simulink model "final_gimbal"  (R2026b)
settings: Solver=ode23t  StopTime=10  MaxStep=max_step  RelTol=1e-4
values from neighbouring files (symbols this model uses):
  kg = SV(i,7)    [servo_dynamics.m]
  m = add_block('simulink/Signal Routing/Mux', sprintf('    [build_model.m]
  N = 0    [LiveView.m]
  s = (1 - a) * B(k, 2:7) + a * B(k+1, 2:7)    [UdpAttitudeSource.m]    (also in build_model.m = solid(mdl, name, 'servo_dummy.stl', color, pos + [90 0 90 0])
  stl = fullfile(fileparts(fileparts(mfilename('fullpath'))), 'cad', 'stl')    [LiveView.m]
undefined symbols (not defined in the file or in its folder): ant_mass, lead_s, log_dt, mount_rate, pwm_rate, q0, servo_mass, SV, t_pure, travel, X, Y, Z
libraries: sm_lib x67, nesl_utility x18
(part 1 of 2)
settings Model: Creator=ruru  LastModifiedBy=ruru
settings SimscapeCC: SimscapeLogType=all  SimscapeNominalValues="[{\"value\":\"1\",\"unit\":\"A\"},{\"value\":\"1\",\"unit\":\"bar\"},{\"value\":\"1\",\"unit\":\"cm^2\"},{\"value\":\"1\",\"unit\":\"cm^3/s\"},{\"value\":\"1\",\"unit\":\"kJ/kg\"},{\"value\":\"1\",\"unit\":\"kW\"},{\"value\":\"1\",\"unit\":\"l\"},{\"value\":\"1\",\"unit\":\"N\"},{\"value\":\"1\",\"unit\":\"N*m\"},{\"value\":\"1\",\"unit\":\"V\"},{\"value\":\"0.001\",\"unit\":\"Wb\"}]"  SimscapeUseEnergyAccounting=off
settings ExplorerConfigSet: SimMechanicsOpenEditorOnUpdate=off

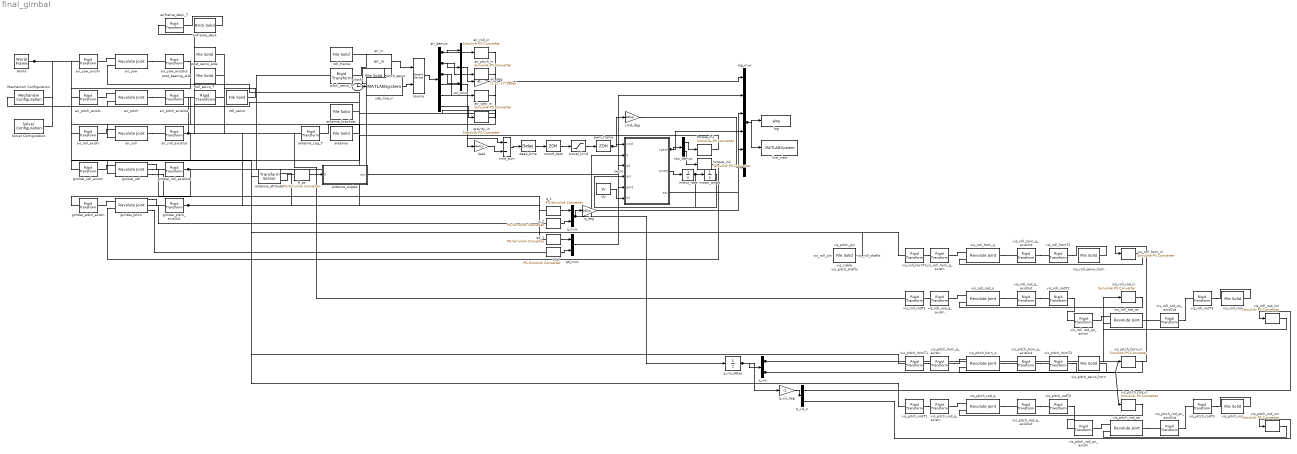
== system final_gimbal ==
  Mechanism Configuration : sm_lib/Utilities/Mechanism Configuration  UniformGravity=TimeVarying  GravityVector=[0 0 -9.80665]  GravityVectorUnits=m/s^2  LinearizationDelta=0.001  JointModeTransitionNonlinearIterations=2
  R_ps : nesl_utility/PS-Simulink Converter  PhysicalDomain=network_engine_domain  SubClassName=ps_output  LeftPortType=input  RightPortType=output  PseudoPeriodic=off  Frequencies=[]  VectorFormat=inherit  Unit=inherit  AffineConversion=off
  SV : Constant  Value=SV
  Solver Configuration : nesl_utility/Solver Configuration  PhysicalDomain=network_engine_domain  SubClassName=solver  LeftPortType=input  RightPortType=generic  Tones=[]  Harmonics=[]  SimulateNoise=off  Profile=off  UseLocalSampling=off  EnableSwitchedLinearOptims=on  FrequencyDomain=off  UseCCode=off  RelTol=0.001  AbsTol=0.001  MinStep=1e-09  ToWorkspace=off  RevertToSquareIcSolve=off  NumHomotopyIterations=100  PhasorMode=off  PhasorModeNumHarmonics=1  ConsistencySolver=NEWTON_XTOL_AFTER_FTOL  CanonicalOrdering=CANONICAL  OptimizeIntermediates=OPTIMIZED  MulticoreSolverChoice=BACKWARD_EULER  IndexReductionMethod=DerivativeReplacement  DoDC=off  ResidualTolerance=1e-09  ConsistencyTolSource=GLOBAL  ConsistencyAbsTol=0.001  ConsistencyRelTol=0.001  ConsistencyTolFactor=0.001  UseLocalSolver=off  LocalSolverChoice=NE_BACKWARD_EULER_ADVANCER  ResolveIndetEquations=on  FunctionEvalNumThread=1  LocalSolverSampleTime=0.001  DoFixedCost=off  MaxNonlinIter=3  MaxModeIter=2  ComputeImpulses=off  ImpulseIterations=2  LinearAlgebra=auto  LinearAlgebraNumThread=0  EquationFormulation=NE_TIME_EF  DelaysMemoryBudget=1024  AutomaticFiltering=on  FilteringTimeConstant=0.001  PartitionStorageMethod=AS_NEEDED  PartitionMemoryBudget=1024  PartitionMethod=BALANCED  MultibodyUseLocalSolver=off  MultibodyLocalSolverChoice=ODE1  MultibodyLocalSolverSampleTime=0.001
  World : sm_lib/Frames and Transforms/World Frame
  air_deg : Gain  Gain=[1 -1 -1]'*180/pi
  air_demux : Demux  Outputs=[1 1 1 2 2 3]
  air_in : FromWorkspace  VariableName=air_in  OutputAfterFinalValue=Holding final value
  air_mux : Mux  Inputs=3
  air_pitch : sm_lib/Joints/Revolute Joint  JointMode=Normal  CompositeWrenchDir=FollowerOnBase  CompositeWrenchFrame=BaseFrame  SenseConstraintForce=off  SenseConstraintTorque=off  SenseTotalForce=off  SenseTotalTorque=off  PositionTargetSpecify=off  PositionTargetPriority=High  PositionTargetValue=0  PositionTargetValueUnits=deg  VelocityTargetSpecify=off  VelocityTargetPriority=High  VelocityTargetValue=0  VelocityTargetValueUnits=deg/s  EquilibriumPosition=0  EquilibriumPositionUnits=deg  SpringStiffness=0  SpringStiffnessUnits=N*m/deg  DampingCoefficient=0  DampingCoefficientUnits=N*m/(deg/s)  LowerLimitSpecify=off  LowerLimitBound=-90  LowerLimitBoundUnits=deg  LowerLimitStiffness=1e4  LowerLimitStiffnessUnits=N*m/deg  LowerLimitDamping=10  LowerLimitDampingUnits=N*m/(deg/s)  LowerLimitTransitionRegionWidth=0.1  LowerLimitTransitionRegionWidthUnits=deg  UpperLimitSpecify=off  UpperLimitBound=90  UpperLimitBoundUnits=deg  UpperLimitStiffness=1e4  UpperLimitStiffnessUnits=N*m/deg  UpperLimitDamping=10  UpperLimitDampingUnits=N*m/(deg/s)  UpperLimitTransitionRegionWidth=0.1  UpperLimitTransitionRegionWidthUnits=deg  TorqueActuationMode=ComputedTorque  MotionActuationMode=InputMotion  SensePosition=off  SenseVelocity=off  SenseAcceleration=off  SenseTorqueForce=off  SenseLowerLimitTorqueForce=off  SenseUpperLimitTorqueForce=off
  air_pitch_axisIn : sm_lib/Frames and Transforms/Rigid Transform  RotationMethod=RotationMatrix  FollAlignAxisA=+X  BaseAlignAxisA=+Y  FollAlignAxisB=+Y  BaseAlignAxisB=+Z  RotationStandardAxis=+Z  RotationAngle=0  RotationAngleUnits=deg  RotationArbitraryAxis=[0 0 1]  RotationSequenceAxes=FollowerAxes  RotationSequence=XYX  RotationSequenceAngles=[0 0 0]  RotationSequenceAnglesUnits=deg  RotationMatrix=[0 1 0;0 0 1;1 0 0]  Quaternion=[1 0 0 0]  TranslationMethod=Cartesian  TranslationCartesianOffset=[0 0 0]  TranslationCartesianOffsetUnits=mm  TranslationStandardAxis=+Z  TranslationStandardOffset=0  TranslationStandardOffsetUnits=m  TranslationROffset=0  TranslationROffsetUnits=m  TranslationThetaOffset=0  TranslationThetaOffsetUnits=deg  TranslationZOffset=0  TranslationZOffsetUnits=m
  air_pitch_axisOut : sm_lib/Frames and Transforms/Rigid Transform  RotationMethod=RotationMatrix  FollAlignAxisA=+X  BaseAlignAxisA=+Y  FollAlignAxisB=+Y  BaseAlignAxisB=+Z  RotationStandardAxis=+Z  RotationAngle=0  RotationAngleUnits=deg  RotationArbitraryAxis=[0 0 1]  RotationSequenceAxes=FollowerAxes  RotationSequence=XYX  RotationSequenceAngles=[0 0 0]  RotationSequenceAnglesUnits=deg  RotationMatrix=[0 0 1;1 0 0;0 1 0]  Quaternion=[1 0 0 0]  TranslationMethod=Cartesian  TranslationCartesianOffset=[0 0 0]  TranslationCartesianOffsetUnits=mm  TranslationStandardAxis=+Z  TranslationStandardOffset=0  TranslationStandardOffsetUnits=m  TranslationROffset=0  TranslationROffsetUnits=m  TranslationThetaOffset=0  TranslationThetaOffsetUnits=deg  TranslationZOffset=0  TranslationZOffsetUnits=m
  air_pitch_in : nesl_utility/Simulink-PS Converter  PhysicalDomain=network_engine_domain  SubClassName=ps_input  LeftPortType=input  RightPortType=output  PseudoPeriodic=off  Frequencies=[]  NoiseDistribution=none  NoiseParameters=[]  Unit=rad  AffineConversion=off  FilteringAndDerivatives=filter  SimscapeFilterOrder=2  InputFilterTimeConstant=air_filter_s  UdotUserProvided=0
  air_roll : sm_lib/Joints/Revolute Joint  JointMode=Normal  CompositeWrenchDir=FollowerOnBase  CompositeWrenchFrame=BaseFrame  SenseConstraintForce=off  SenseConstraintTorque=off  SenseTotalForce=off  SenseTotalTorque=off  PositionTargetSpecify=off  PositionTargetPriority=High  PositionTargetValue=0  PositionTargetValueUnits=deg  VelocityTargetSpecify=off  VelocityTargetPriority=High  VelocityTargetValue=0  VelocityTargetValueUnits=deg/s  EquilibriumPosition=0  EquilibriumPositionUnits=deg  SpringStiffness=0  SpringStiffnessUnits=N*m/deg  DampingCoefficient=0  DampingCoefficientUnits=N*m/(deg/s)  LowerLimitSpecify=off  LowerLimitBound=-90  LowerLimitBoundUnits=deg  LowerLimitStiffness=1e4  LowerLimitStiffnessUnits=N*m/deg  LowerLimitDamping=10  LowerLimitDampingUnits=N*m/(deg/s)  LowerLimitTransitionRegionWidth=0.1  LowerLimitTransitionRegionWidthUnits=deg  UpperLimitSpecify=off  UpperLimitBound=90  UpperLimitBoundUnits=deg  UpperLimitStiffness=1e4  UpperLimitStiffnessUnits=N*m/deg  UpperLimitDamping=10  UpperLimitDampingUnits=N*m/(deg/s)  UpperLimitTransitionRegionWidth=0.1  UpperLimitTransitionRegionWidthUnits=deg  TorqueActuationMode=ComputedTorque  MotionActuationMode=InputMotion  SensePosition=off  SenseVelocity=off  SenseAcceleration=off  SenseTorqueForce=off  SenseLowerLimitTorqueForce=off  SenseUpperLimitTorqueForce=off
  air_roll_axisIn : sm_lib/Frames and Transforms/Rigid Transform  RotationMethod=RotationMatrix  FollAlignAxisA=+X  BaseAlignAxisA=+Y  FollAlignAxisB=+Y  BaseAlignAxisB=+Z  RotationStandardAxis=+Z  RotationAngle=0  RotationAngleUnits=deg  RotationArbitraryAxis=[0 0 1]  RotationSequenceAxes=FollowerAxes  RotationSequence=XYX  RotationSequenceAngles=[0 0 0]  RotationSequenceAnglesUnits=deg  RotationMatrix=[0 0 1;1 0 0;0 1 0]  Quaternion=[1 0 0 0]  TranslationMethod=Cartesian  TranslationCartesianOffset=[0 0 0]  TranslationCartesianOffsetUnits=mm  TranslationStandardAxis=+Z  TranslationStandardOffset=0  TranslationStandardOffsetUnits=m  TranslationROffset=0  TranslationROffsetUnits=m  TranslationThetaOffset=0  TranslationThetaOffsetUnits=deg  TranslationZOffset=0  TranslationZOffsetUnits=m
  air_roll_axisOut : sm_lib/Frames and Transforms/Rigid Transform  RotationMethod=RotationMatrix  FollAlignAxisA=+X  BaseAlignAxisA=+Y  FollAlignAxisB=+Y  BaseAlignAxisB=+Z  RotationStandardAxis=+Z  RotationAngle=0  RotationAngleUnits=deg  RotationArbitraryAxis=[0 0 1]  RotationSequenceAxes=FollowerAxes  RotationSequence=XYX  RotationSequenceAngles=[0 0 0]  RotationSequenceAnglesUnits=deg  RotationMatrix=[0 1 0;0 0 1;1 0 0]  Quaternion=[1 0 0 0]  TranslationMethod=Cartesian  TranslationCartesianOffset=[0 0 0]  TranslationCartesianOffsetUnits=mm  TranslationStandardAxis=+Z  TranslationStandardOffset=0  TranslationStandardOffsetUnits=m  TranslationROffset=0  TranslationROffsetUnits=m  TranslationThetaOffset=0  TranslationThetaOffsetUnits=deg  TranslationZOffset=0  TranslationZOffsetUnits=m
  air_roll_in : nesl_utility/Simulink-PS Converter  PhysicalDomain=network_engine_domain  SubClassName=ps_input  LeftPortType=input  RightPortType=output  PseudoPeriodic=off  Frequencies=[]  NoiseDistribution=none  NoiseParameters=[]  Unit=rad  AffineConversion=off  FilteringAndDerivatives=filter  SimscapeFilterOrder=2  InputFilterTimeConstant=air_filter_s  UdotUserProvided=0
  air_yaw : sm_lib/Joints/Revolute Joint  JointMode=Normal  CompositeWrenchDir=FollowerOnBase  CompositeWrenchFrame=BaseFrame  SenseConstraintForce=off  SenseConstraintTorque=off  SenseTotalForce=off  SenseTotalTorque=off  PositionTargetSpecify=off  PositionTargetPriority=High  PositionTargetValue=0  PositionTargetValueUnits=deg  VelocityTargetSpecify=off  VelocityTargetPriority=High  VelocityTargetValue=0  VelocityTargetValueUnits=deg/s  EquilibriumPosition=0  EquilibriumPositionUnits=deg  SpringStiffness=0  SpringStiffnessUnits=N*m/deg  DampingCoefficient=0  DampingCoefficientUnits=N*m/(deg/s)  LowerLimitSpecify=off  LowerLimitBound=-90  LowerLimitBoundUnits=deg  LowerLimitStiffness=1e4  LowerLimitStiffnessUnits=N*m/deg  LowerLimitDamping=10  LowerLimitDampingUnits=N*m/(deg/s)  LowerLimitTransitionRegionWidth=0.1  LowerLimitTransitionRegionWidthUnits=deg  UpperLimitSpecify=off  UpperLimitBound=90  UpperLimitBoundUnits=deg  UpperLimitStiffness=1e4  UpperLimitStiffnessUnits=N*m/deg  UpperLimitDamping=10  UpperLimitDampingUnits=N*m/(deg/s)  UpperLimitTransitionRegionWidth=0.1  UpperLimitTransitionRegionWidthUnits=deg  TorqueActuationMode=ComputedTorque  MotionActuationMode=InputMotion  SensePosition=off  SenseVelocity=off  SenseAcceleration=off  SenseTorqueForce=off  SenseLowerLimitTorqueForce=off  SenseUpperLimitTorqueForce=off
  air_yaw_axisIn : sm_lib/Frames and Transforms/Rigid Transform  RotationMethod=RotationMatrix  FollAlignAxisA=+X  BaseAlignAxisA=+Y  FollAlignAxisB=+Y  BaseAlignAxisB=+Z  RotationStandardAxis=+Z  RotationAngle=0  RotationAngleUnits=deg  RotationArbitraryAxis=[0 0 1]  RotationSequenceAxes=FollowerAxes  RotationSequence=XYX  RotationSequenceAngles=[0 0 0]  RotationSequenceAnglesUnits=deg  RotationMatrix=[1 0 0;0 1 0;0 0 1]  Quaternion=[1 0 0 0]  TranslationMethod=Cartesian  TranslationCartesianOffset=[0 0 0]  TranslationCartesianOffsetUnits=mm  TranslationStandardAxis=+Z  TranslationStandardOffset=0  TranslationStandardOffsetUnits=m  TranslationROffset=0  TranslationROffsetUnits=m  TranslationThetaOffset=0  TranslationThetaOffsetUnits=deg  TranslationZOffset=0  TranslationZOffsetUnits=m
  air_yaw_axisOut : sm_lib/Frames and Transforms/Rigid Transform  RotationMethod=RotationMatrix  FollAlignAxisA=+X  BaseAlignAxisA=+Y  FollAlignAxisB=+Y  BaseAlignAxisB=+Z  RotationStandardAxis=+Z  RotationAngle=0  RotationAngleUnits=deg  RotationArbitraryAxis=[0 0 1]  RotationSequenceAxes=FollowerAxes  RotationSequence=XYX  RotationSequenceAngles=[0 0 0]  RotationSequenceAnglesUnits=deg  RotationMatrix=[1 0 0;0 1 0;0 0 1]  Quaternion=[1 0 0 0]  TranslationMethod=Cartesian  TranslationCartesianOffset=[0 0 0]  TranslationCartesianOffsetUnits=mm  TranslationStandardAxis=+Z  TranslationStandardOffset=0  TranslationStandardOffsetUnits=m  TranslationROffset=0  TranslationROffsetUnits=m  TranslationThetaOffset=0  TranslationThetaOffsetUnits=deg  TranslationZOffset=0  TranslationZOffsetUnits=m
  air_yaw_in : nesl_utility/Simulink-PS Converter  PhysicalDomain=network_engine_domain  SubClassName=ps_input  LeftPortType=input  RightPortType=output  PseudoPeriodic=off  Frequencies=[]  NoiseDistribution=none  NoiseParameters=[]  Unit=rad  AffineConversion=off  FilteringAndDerivatives=filter  SimscapeFilterOrder=2  InputFilterTimeConstant=air_filter_s  UdotUserProvided=0
  airframe_deck : sm_lib/Body Elements/Brick Solid  BrickDimensions=[0.7 0.5 0.004]  BrickDimensionsUnits=m  ExportEntireGeometry=off  InertiaType=CalculateFromGeometry  BasedOnType=Density  Density=1000  DensityUnits=kg/m^3  Mass=1  MassUnits=kg  CenterOfMass=[0 0 0]  CenterOfMassUnits=m  MomentsOfInertia=[1 1 1]  MomentsOfInertiaUnits=kg*m^2  ProductsOfInertia=[0 0 0]  ProductsOfInertiaUnits=kg*m^2  GraphicType=FromGeometry  MarkerShape=Sphere  MarkerSize=10  GraphicVisPropType=SimpleVisualProperties  GraphicDiffuseColor=[0.8 0.8 0.78]  GraphicOpacity=1  GraphicSpecularColor=[0.5 0.5 0.5 1.0]  GraphicAmbientColor=[0.15 0.15 0.15 1.0]  GraphicEmissiveColor=[0.0 0.0 0.0 1.0]  GraphicShininess=75  DoExposeReferenceFrame=on  SerializedFrames=<Frames/>
  airframe_deck_T : sm_lib/Frames and Transforms/Rigid Transform  RotationMethod=RotationMatrix  FollAlignAxisA=+X  BaseAlignAxisA=+Y  FollAlignAxisB=+Y  BaseAlignAxisB=+Z  RotationStandardAxis=+Z  RotationAngle=0  RotationAngleUnits=deg  RotationArbitraryAxis=[0 0 1]  RotationSequenceAxes=FollowerAxes  RotationSequence=XYX  RotationSequenceAngles=[0 0 0]  RotationSequenceAnglesUnits=deg  RotationMatrix=[1 0 0;0 1 0;0 0 1]  Quaternion=[1 0 0 0]  TranslationMethod=Cartesian  TranslationCartesianOffset=[0 0 -192]  TranslationCartesianOffsetUnits=mm  TranslationStandardAxis=+Z  TranslationStandardOffset=0  TranslationStandardOffsetUnits=m  TranslationROffset=0  TranslationROffsetUnits=m  TranslationThetaOffset=0  TranslationThetaOffsetUnits=deg  TranslationZOffset=0  TranslationZOffsetUnits=m
  antenna : sm_lib/Body Elements/File Solid  ExtGeomFileName=/Users/ruru/Documenti-local/projects/hackathon/edth/hackathon-paris-2026/cad/stl/antenna_crpa_d370.stl  UnitType=Custom  ExtGeomFileUnits=mm  StepReaderType=HEX  ExportConvexHullGeometry=off  InertiaType=CalculateFromGeometry  BasedOnType=Mass  Density=1000  DensityUnits=kg/m^3  Mass=ant_mass  MassUnits=kg  CenterOfMass=[0 0 0]  CenterOfMassUnits=m  MomentsOfInertia=[1 1 1]  MomentsOfInertiaUnits=kg*m^2  ProductsOfInertia=[0 0 0]  ProductsOfInertiaUnits=kg*m^2  GraphicType=FromGeometry  MarkerShape=Sphere  MarkerSize=10  GraphicVisPropType=SimpleVisualProperties  GraphicDiffuseColor=[0.9 0.91 0.92]  GraphicOpacity=0.55  GraphicSpecularColor=[0.5 0.5 0.5 1.0]  GraphicAmbientColor=[0.15 0.15 0.15 1.0]  GraphicEmissiveColor=[0.0 0.0 0.0 1.0]  GraphicShininess=75  DoExposeReferenceFrame=on  SerializedFrames=<Frames/>
  antenna_angles : MATLAB Function  TreatAsAtomicUnit=on
  antenna_attitude : sm_lib/Frames and Transforms/Transform Sensor  ObservationFrame=World  ExpressedInFrame=World  RotationSequence=XYX  SenseAngle=off  SenseAxis=off  SenseQ=off  SenseR=on  SenseRotationSequence=off  SenseOmegaX=off  SenseOmegaY=off  SenseOmegaZ=off  SenseOmega=off  SenseQDot=off  SenseRDot=off  SenseRotationSequenceDot=off  SenseAlphaX=off  SenseAlphaY=off  SenseAlphaZ=off  SenseAlpha=off  SenseQDDot=off  SenseRDDot=off  SenseX=off  SenseY=off  SenseZ=off  SenseXYZ=off  SenseRad=off  SenseAzim=off  SenseDist=off  SenseInc=off  SenseXDot=off  SenseYDot=off  SenseZDot=off  SenseXYZDot=off  SenseRadDot=off  SenseAzimDot=off  SenseDistDot=off  SenseIncDot=off  SenseXDDot=off  SenseYDDot=off  SenseZDDot=off  SenseXYZDDot=off  SenseRadDDot=off  SenseAzimDDot=off  SenseDistDDot=off  SenseIncDDot=off
  antenna_brackets : sm_lib/Body Elements/File Solid  ExtGeomFileName=/Users/ruru/Documenti-local/projects/hackathon/edth/hackathon-paris-2026/cad/stl/antenna_brackets.stl  UnitType=Custom  ExtGeomFileUnits=mm  StepReaderType=HEX  ExportConvexHullGeometry=off  InertiaType=CalculateFromGeometry  BasedOnType=Density  Density=rho_struct  DensityUnits=kg/m^3  Mass=1  MassUnits=kg  CenterOfMass=[0 0 0]  CenterOfMassUnits=m  MomentsOfInertia=[1 1 1]  MomentsOfInertiaUnits=kg*m^2  ProductsOfInertia=[0 0 0]  ProductsOfInertiaUnits=kg*m^2  GraphicType=FromGeometry  MarkerShape=Sphere  MarkerSize=10  GraphicVisPropType=SimpleVisualProperties  GraphicDiffuseColor=[0.02 0.59 0.41]  GraphicOpacity=1  GraphicSpecularColor=[0.5 0.5 0.5 1.0]  GraphicAmbientColor=[0.15 0.15 0.15 1.0]  GraphicEmissiveColor=[0.0 0.0 0.0 1.0]  GraphicShininess=75  DoExposeReferenceFrame=on  SerializedFrames=<Frames/>
  antenna_cog_T : sm_lib/Frames and Transforms/Rigid Transform  RotationMethod=None  FollAlignAxisA=+X  BaseAlignAxisA=+Y  FollAlignAxisB=+Y  BaseAlignAxisB=+Z  RotationStandardAxis=+Z  RotationAngle=0  RotationAngleUnits=deg  RotationArbitraryAxis=[0 0 1]  RotationSequenceAxes=FollowerAxes  RotationSequence=XYX  RotationSequenceAngles=[0 0 0]  RotationSequenceAnglesUnits=deg  RotationMatrix=[1 0 0;0 1 0;0 0 1]  Quaternion=[1 0 0 0]  TranslationMethod=Cartesian  TranslationCartesianOffset=cog_offset_mm  TranslationCartesianOffsetUnits=mm  TranslationStandardAxis=+Z  TranslationStandardOffset=0  TranslationStandardOffsetUnits=m  TranslationROffset=0  TranslationROffsetUnits=m  TranslationThetaOffset=0  TranslationThetaOffsetUnits=deg  TranslationZOffset=0  TranslationZOffsetUnits=m
  clock : Clock
  cmd_deg : Gain  Gain=180/pi
  cmd_sum : Sum  Inputs=--
  dead_time : TransportDelay  DelayTime=t_pure  InitialOutput=q0
  gimbal_pitch : sm_lib/Joints/Revolute Joint  JointMode=Normal  CompositeWrenchDir=FollowerOnBase  CompositeWrenchFrame=BaseFrame  SenseConstraintForce=off  SenseConstraintTorque=off  SenseTotalForce=off  SenseTotalTorque=off  PositionTargetSpecify=on  PositionTargetPriority=High  PositionTargetValue=q0(2)  PositionTargetValueUnits=rad  VelocityTargetSpecify=off  VelocityTargetPriority=High  VelocityTargetValue=0  VelocityTargetValueUnits=deg/s  EquilibriumPosition=0  EquilibriumPositionUnits=deg  SpringStiffness=cable_k  SpringStiffnessUnits=N*m/rad  DampingCoefficient=bearing_b  DampingCoefficientUnits=N*m*s/rad  LowerLimitSpecify=off  LowerLimitBound=-90  LowerLimitBoundUnits=deg  LowerLimitStiffness=1e4  LowerLimitStiffnessUnits=N*m/deg  LowerLimitDamping=10  LowerLimitDampingUnits=N*m/(deg/s)  LowerLimitTransitionRegionWidth=0.1  LowerLimitTransitionRegionWidthUnits=deg  UpperLimitSpecify=off  UpperLimitBound=90  UpperLimitBoundUnits=deg  UpperLimitStiffness=1e4  UpperLimitStiffnessUnits=N*m/deg  UpperLimitDamping=10  UpperLimitDampingUnits=N*m/(deg/s)  UpperLimitTransitionRegionWidth=0.1  UpperLimitTransitionRegionWidthUnits=deg  TorqueActuationMode=InputTorque  MotionActuationMode=ComputedMotion  SensePosition=on  SenseVelocity=on  SenseAcceleration=off  SenseTorqueForce=off  SenseLowerLimitTorqueForce=off  SenseUpperLimitTorqueForce=off
  gimbal_pitch_axisIn : sm_lib/Frames and Transforms/Rigid Transform  RotationMethod=RotationMatrix  FollAlignAxisA=+X  BaseAlignAxisA=+Y  FollAlignAxisB=+Y  BaseAlignAxisB=+Z  RotationStandardAxis=+Z  RotationAngle=0  RotationAngleUnits=deg  RotationArbitraryAxis=[0 0 1]  RotationSequenceAxes=FollowerAxes  RotationSequence=XYX  RotationSequenceAngles=[0 0 0]  RotationSequenceAnglesUnits=deg  RotationMatrix=[0 1 0;0 0 1;1 0 0]  Quaternion=[1 0 0 0]  TranslationMethod=Cartesian  TranslationCartesianOffset=[0 0 0]  TranslationCartesianOffsetUnits=mm  TranslationStandardAxis=+Z  TranslationStandardOffset=0  TranslationStandardOffsetUnits=m  TranslationROffset=0  TranslationROffsetUnits=m  TranslationThetaOffset=0  TranslationThetaOffsetUnits=deg  TranslationZOffset=0  TranslationZOffsetUnits=m
  gimbal_pitch_axisOut : sm_lib/Frames and Transforms/Rigid Transform  RotationMethod=RotationMatrix  FollAlignAxisA=+X  BaseAlignAxisA=+Y  FollAlignAxisB=+Y  BaseAlignAxisB=+Z  RotationStandardAxis=+Z  RotationAngle=0  RotationAngleUnits=deg  RotationArbitraryAxis=[0 0 1]  RotationSequenceAxes=FollowerAxes  RotationSequence=XYX  RotationSequenceAngles=[0 0 0]  RotationSequenceAnglesUnits=deg  RotationMatrix=[0 0 1;1 0 0;0 1 0]  Quaternion=[1 0 0 0]  TranslationMethod=Cartesian  TranslationCartesianOffset=[0 0 0]  TranslationCartesianOffsetUnits=mm  TranslationStandardAxis=+Z  TranslationStandardOffset=0  TranslationStandardOffsetUnits=m  TranslationROffset=0  TranslationROffsetUnits=m  TranslationThetaOffset=0  TranslationThetaOffsetUnits=deg  TranslationZOffset=0  TranslationZOffsetUnits=m
  gimbal_roll : sm_lib/Joints/Revolute Joint  JointMode=Normal  CompositeWrenchDir=FollowerOnBase  CompositeWrenchFrame=BaseFrame  SenseConstraintForce=off  SenseConstraintTorque=off  SenseTotalForce=off  SenseTotalTorque=off  PositionTargetSpecify=on  PositionTargetPriority=High  PositionTargetValue=q0(1)  PositionTargetValueUnits=rad  VelocityTargetSpecify=off  VelocityTargetPriority=High  VelocityTargetValue=0  VelocityTargetValueUnits=deg/s  EquilibriumPosition=0  EquilibriumPositionUnits=deg  SpringStiffness=cable_k  SpringStiffnessUnits=N*m/rad  DampingCoefficient=bearing_b  DampingCoefficientUnits=N*m*s/rad  LowerLimitSpecify=off  LowerLimitBound=-90  LowerLimitBoundUnits=deg  LowerLimitStiffness=1e4  LowerLimitStiffnessUnits=N*m/deg  LowerLimitDamping=10  LowerLimitDampingUnits=N*m/(deg/s)  LowerLimitTransitionRegionWidth=0.1  LowerLimitTransitionRegionWidthUnits=deg  UpperLimitSpecify=off  UpperLimitBound=90  UpperLimitBoundUnits=deg  UpperLimitStiffness=1e4  UpperLimitStiffnessUnits=N*m/deg  UpperLimitDamping=10  UpperLimitDampingUnits=N*m/(deg/s)  UpperLimitTransitionRegionWidth=0.1  UpperLimitTransitionRegionWidthUnits=deg  TorqueActuationMode=InputTorque  MotionActuationMode=ComputedMotion  SensePosition=on  SenseVelocity=on  SenseAcceleration=off  SenseTorqueForce=off  SenseLowerLimitTorqueForce=off  SenseUpperLimitTorqueForce=off
  gimbal_roll_axisIn : sm_lib/Frames and Transforms/Rigid Transform  RotationMethod=RotationMatrix  FollAlignAxisA=+X  BaseAlignAxisA=+Y  FollAlignAxisB=+Y  BaseAlignAxisB=+Z  RotationStandardAxis=+Z  RotationAngle=0  RotationAngleUnits=deg  RotationArbitraryAxis=[0 0 1]  RotationSequenceAxes=FollowerAxes  RotationSequence=XYX  RotationSequenceAngles=[0 0 0]  RotationSequenceAnglesUnits=deg  RotationMatrix=[0 0 1;1 0 0;0 1 0]  Quaternion=[1 0 0 0]  TranslationMethod=Cartesian  TranslationCartesianOffset=[0 0 0]  TranslationCartesianOffsetUnits=mm  TranslationStandardAxis=+Z  TranslationStandardOffset=0  TranslationStandardOffsetUnits=m  TranslationROffset=0  TranslationROffsetUnits=m  TranslationThetaOffset=0  TranslationThetaOffsetUnits=deg  TranslationZOffset=0  TranslationZOffsetUnits=m
  gimbal_roll_axisOut : sm_lib/Frames and Transforms/Rigid Transform  RotationMethod=RotationMatrix  FollAlignAxisA=+X  BaseAlignAxisA=+Y  FollAlignAxisB=+Y  BaseAlignAxisB=+Z  RotationStandardAxis=+Z  RotationAngle=0  RotationAngleUnits=deg  RotationArbitraryAxis=[0 0 1]  RotationSequenceAxes=FollowerAxes  RotationSequence=XYX  RotationSequenceAngles=[0 0 0]  RotationSequenceAnglesUnits=deg  RotationMatrix=[0 1 0;0 0 1;1 0 0]  Quaternion=[1 0 0 0]  TranslationMethod=Cartesian  TranslationCartesianOffset=[0 0 0]  TranslationCartesianOffsetUnits=mm  TranslationStandardAxis=+Z  TranslationStandardOffset=0  TranslationStandardOffsetUnits=m  TranslationROffset=0  TranslationROffsetUnits=m  TranslationThetaOffset=0  TranslationThetaOffsetUnits=deg  TranslationZOffset=0  TranslationZOffsetUnits=m
  gravity_in : nesl_utility/Simulink-PS Converter  PhysicalDomain=network_engine_domain  SubClassName=ps_input  LeftPortType=input  RightPortType=output  PseudoPeriodic=off  Frequencies=[]  NoiseDistribution=none  NoiseParameters=[]  Unit=m/s^2  AffineConversion=off  FilteringAndDerivatives=provide  SimscapeFilterOrder=1  InputFilterTimeConstant=0.001  UdotUserProvided=0
  lead : Gain  Gain=lead_s
  live_view : MATLABSystem  System=LiveView  Window=20  Show=true  SimulateUsing=Interpreted execution
      mask Type: LiveView
  log : ToWorkspace  VariableName=glog  SampleTime=log_dt
  log_mux : Mux  Inputs=6
  motor_angle : Integrator  InitialCondition=q0
  motor_rate : Integrator  InitialCondition=[0;0]
  mount_task : ZeroOrderHold  SampleTime=1/mount_rate
  pitch_servo : sm_lib/Body Elements/File Solid  ExtGeomFileName=/Users/ruru/Documenti-local/projects/hackathon/edth/hackathon-paris-2026/cad/stl/servo_dummy.stl  UnitType=Custom  ExtGeomFileUnits=mm  StepReaderType=HEX  ExportConvexHullGeometry=off  InertiaType=CalculateFromGeometry  BasedOnType=Mass  Density=1000  DensityUnits=kg/m^3  Mass=servo_mass  MassUnits=kg  CenterOfMass=[0 0 0]  CenterOfMassUnits=m  MomentsOfInertia=[1 1 1]  MomentsOfInertiaUnits=kg*m^2  ProductsOfInertia=[0 0 0]  ProductsOfInertiaUnits=kg*m^2  GraphicType=FromGeometry  MarkerShape=Sphere  MarkerSize=10  GraphicVisPropType=SimpleVisualProperties  GraphicDiffuseColor=[0.12 0.16 0.22]  GraphicOpacity=1  GraphicSpecularColor=[0.5 0.5 0.5 1.0]  GraphicAmbientColor=[0.15 0.15 0.15 1.0]  GraphicEmissiveColor=[0.0 0.0 0.0 1.0]  GraphicShininess=75  DoExposeReferenceFrame=on  SerializedFrames=<Frames/>
  pitch_servo_T : sm_lib/Frames and Transforms/Rigid Transform  RotationMethod=RotationMatrix  FollAlignAxisA=+X  BaseAlignAxisA=+Y  FollAlignAxisB=+Y  BaseAlignAxisB=+Z  RotationStandardAxis=+Z  RotationAngle=0  RotationAngleUnits=deg  RotationArbitraryAxis=[0 0 1]  RotationSequenceAxes=FollowerAxes  RotationSequence=XYX  RotationSequenceAngles=[0 0 0]  RotationSequenceAnglesUnits=deg  RotationMatrix=[1 0 0;0 0 1;0 -1 0]  Quaternion=[1 0 0 0]  TranslationMethod=Cartesian  TranslationCartesianOffset=[140 189 0]  TranslationCartesianOffsetUnits=mm  TranslationStandardAxis=+Z  TranslationStandardOffset=0  TranslationStandardOffsetUnits=m  TranslationROffset=0  TranslationROffsetUnits=m  TranslationThetaOffset=0  TranslationThetaOffsetUnits=deg  TranslationZOffset=0  TranslationZOffsetUnits=m
  post_bearing_side : sm_lib/Body Elements/File Solid  ExtGeomFileName=/Users/ruru/Documenti-local/projects/hackathon/edth/hackathon-paris-2026/cad/stl/post_bearing_side.stl  UnitType=Custom  ExtGeomFileUnits=mm  StepReaderType=HEX  ExportConvexHullGeometry=off  InertiaType=CalculateFromGeometry  BasedOnType=Density  Density=rho_struct  DensityUnits=kg/m^3  Mass=1  MassUnits=kg  CenterOfMass=[0 0 0]  CenterOfMassUnits=m  MomentsOfInertia=[1 1 1]  MomentsOfInertiaUnits=kg*m^2  ProductsOfInertia=[0 0 0]  ProductsOfInertiaUnits=kg*m^2  GraphicType=FromGeometry  MarkerShape=Sphere  MarkerSize=10  GraphicVisPropType=SimpleVisualProperties  GraphicDiffuseColor=[0.42 0.45 0.5]  GraphicOpacity=1  GraphicSpecularColor=[0.5 0.5 0.5 1.0]  GraphicAmbientColor=[0.15 0.15 0.15 1.0]  GraphicEmissiveColor=[0.0 0.0 0.0 1.0]  GraphicShininess=75  DoExposeReferenceFrame=on  SerializedFrames=<Frames/>
  post_servo_side : sm_lib/Body Elements/File Solid  ExtGeomFileName=/Users/ruru/Documenti-local/projects/hackathon/edth/hackathon-paris-2026/cad/stl/post_servo_side.stl  UnitType=Custom  ExtGeomFileUnits=mm  StepReaderType=HEX  ExportConvexHullGeometry=off  InertiaType=CalculateFromGeometry  BasedOnType=Density  Density=rho_struct  DensityUnits=kg/m^3  Mass=1  MassUnits=kg  CenterOfMass=[0 0 0]  CenterOfMassUnits=m  MomentsOfInertia=[1 1 1]  MomentsOfInertiaUnits=kg*m^2  ProductsOfInertia=[0 0 0]  ProductsOfInertiaUnits=kg*m^2  GraphicType=FromGeometry  MarkerShape=Sphere  MarkerSize=10  GraphicVisPropType=SimpleVisualProperties  GraphicDiffuseColor=[0.42 0.45 0.5]  GraphicOpacity=1  GraphicSpecularColor=[0.5 0.5 0.5 1.0]  GraphicAmbientColor=[0.15 0.15 0.15 1.0]  GraphicEmissiveColor=[0.0 0.0 0.0 1.0]  GraphicShininess=75  DoExposeReferenceFrame=on  SerializedFrames=<Frames/>
  pwm_frame : ZeroOrderHold  SampleTime=1/pwm_rate
  q_1 : nesl_utility/PS-Simulink Converter  PhysicalDomain=network_engine_domain  SubClassName=ps_output  LeftPortType=input  RightPortType=output  PseudoPeriodic=off  Frequencies=[]  VectorFormat=inherit  Unit=rad  AffineConversion=off
  q_2 : nesl_utility/PS-Simulink Converter  PhysicalDomain=network_engine_domain  SubClassName=ps_output  LeftPortType=input  RightPortType=output  PseudoPeriodic=off  Frequencies=[]  VectorFormat=inherit  Unit=rad  AffineConversion=off
  q_deg : Gain  Gain=180/pi
  q_mux : Mux  Inputs=2
  q_vis : Demux  Outputs=2
  q_vis_delay : UnitDelay  InitialCondition=q0  SampleTime=0.005
  q_vis_n : Demux  Outputs=2
  q_vis_neg : Gain  Gain=-1
  qd_1 : nesl_utility/PS-Simulink Converter  PhysicalDomain=network_engine_domain  SubClassName=ps_output  LeftPortType=input  RightPortType=output  PseudoPeriodic=off  Frequencies=[]  VectorFormat=inherit  Unit=rad/s  AffineConversion=off
  qd_2 : nesl_utility/PS-Simulink Converter  PhysicalDomain=network_engine_domain  SubClassName=ps_output  LeftPortType=input  RightPortType=output  PseudoPeriodic=off  Frequencies=[]  VectorFormat=inherit  Unit=rad/s  AffineConversion=off
  qd_mux : Mux  Inputs=2
  roll_frame : sm_lib/Body Elements/File Solid  ExtGeomFileName=/Users/ruru/Documenti-local/projects/hackathon/edth/hackathon-paris-2026/cad/stl/roll_frame.stl  UnitType=Custom  ExtGeomFileUnits=mm  StepReaderType=HEX  ExportConvexHullGeometry=off  InertiaType=CalculateFromGeometry  BasedOnType=Density  Density=rho_struct  DensityUnits=kg/m^3  Mass=1  MassUnits=kg  CenterOfMass=[0 0 0]  CenterOfMassUnits=m  MomentsOfInertia=[1 1 1]  MomentsOfInertiaUnits=kg*m^2  ProductsOfInertia=[0 0 0]  ProductsOfInertiaUnits=kg*m^2  GraphicType=FromGeometry  MarkerShape=Sphere  MarkerSize=10  GraphicVisPropType=SimpleVisualProperties  GraphicDiffuseColor=[0.15 0.39 0.92]  GraphicOpacity=1  GraphicSpecularColor=[0.5 0.5 0.5 1.0]  GraphicAmbientColor=[0.15 0.15 0.15 1.0]  GraphicEmissiveColor=[0.0 0.0 0.0 1.0]  GraphicShininess=75  DoExposeReferenceFrame=on  SerializedFrames=<Frames/>
  roll_servo : sm_lib/Body Elements/File Solid  ExtGeomFileName=/Users/ruru/Documenti-local/projects/hackathon/edth/hackathon-paris-2026/cad/stl/servo_dummy.stl  UnitType=Custom  ExtGeomFileUnits=mm  StepReaderType=HEX  ExportConvexHullGeometry=off  InertiaType=CalculateFromGeometry  BasedOnType=Mass  Density=1000  DensityUnits=kg/m^3  Mass=servo_mass  MassUnits=kg  CenterOfMass=[0 0 0]  CenterOfMassUnits=m  MomentsOfInertia=[1 1 1]  MomentsOfInertiaUnits=kg*m^2  ProductsOfInertia=[0 0 0]  ProductsOfInertiaUnits=kg*m^2  GraphicType=FromGeometry  MarkerShape=Sphere  MarkerSize=10  GraphicVisPropType=SimpleVisualProperties  GraphicDiffuseColor=[0.12 0.16 0.22]  GraphicOpacity=1  GraphicSpecularColor=[0.5 0.5 0.5 1.0]  GraphicAmbientColor=[0.15 0.15 0.15 1.0]  GraphicEmissiveColor=[0.0 0.0 0.0 1.0]  GraphicShininess=75  DoExposeReferenceFrame=on  SerializedFrames=<Frames/>
  roll_servo_T : sm_lib/Frames and Transforms/Rigid Transform  RotationMethod=RotationMatrix  FollAlignAxisA=+X  BaseAlignAxisA=+Y  FollAlignAxisB=+Y  BaseAlignAxisB=+Z  RotationStandardAxis=+Z  RotationAngle=0  RotationAngleUnits=deg  RotationArbitraryAxis=[0 0 1]  RotationSequenceAxes=FollowerAxes  RotationSequence=XYX  RotationSequenceAngles=[0 0 0]  RotationSequenceAnglesUnits=deg  RotationMatrix=[0 0 1;0 1 0;-1 0 0]  Quaternion=[1 0 0 0]  TranslationMethod=Cartesian  TranslationCartesianOffset=[188 0 -127]  TranslationCartesianOffsetUnits=mm  TranslationStandardAxis=+Z  TranslationStandardOffset=0  TranslationStandardOffsetUnits=m  TranslationROffset=0  TranslationROffsetUnits=m  TranslationThetaOffset=0  TranslationThetaOffsetUnits=deg  TranslationZOffset=0  TranslationZOffsetUnits=m
  servo : MATLAB Function  TreatAsAtomicUnit=on
  source : VariantSource  VariantControls={LIVE==0, LIVE==1}
  tau_demux : Demux  Outputs=2
  torque_in1 : nesl_utility/Simulink-PS Converter  PhysicalDomain=network_engine_domain  SubClassName=ps_input  LeftPortType=input  RightPortType=output  PseudoPeriodic=off  Frequencies=[]  NoiseDistribution=none  NoiseParameters=[]  Unit=N*m  AffineConversion=off  FilteringAndDerivatives=provide  SimscapeFilterOrder=1  InputFilterTimeConstant=0.001  UdotUserProvided=0
  torque_in2 : nesl_utility/Simulink-PS Converter  PhysicalDomain=network_engine_domain  SubClassName=ps_input  LeftPortType=input  RightPortType=output  PseudoPeriodic=off  Frequencies=[]  NoiseDistribution=none  NoiseParameters=[]  Unit=N*m  AffineConversion=off  FilteringAndDerivatives=provide  SimscapeFilterOrder=1  InputFilterTimeConstant=0.001  UdotUserProvided=0
  travel_limit : Saturate  UpperLimit=travel  LowerLimit=-travel
  udp_live_in : MATLABSystem  System=UdpAttitudeSource  Port=9870  Lag=0.06  SimulateUsing=Interpreted execution
      mask Type: UdpAttitudeSource
  vis_cable : sm_lib/Body Elements/File Solid  ExtGeomFileName=/Users/ruru/Documenti-local/projects/hackathon/edth/hackathon-paris-2026/cad/stl/cable_dummy.stl  UnitType=Custom  ExtGeomFileUnits=mm  StepReaderType=HEX  ExportConvexHullGeometry=off  InertiaType=CalculateFromGeometry  BasedOnType=Mass  Density=1000  DensityUnits=kg/m^3  Mass=1e-6  MassUnits=kg  CenterOfMass=[0 0 0]  CenterOfMassUnits=m  MomentsOfInertia=[1 1 1]  MomentsOfInertiaUnits=kg*m^2  ProductsOfInertia=[0 0 0]  ProductsOfInertiaUnits=kg*m^2  GraphicType=FromGeometry  MarkerShape=Sphere  MarkerSize=10  GraphicVisPropType=SimpleVisualProperties  GraphicDiffuseColor=[0.49 0.23 0.93]  GraphicOpacity=1  GraphicSpecularColor=[0.5 0.5 0.5 1.0]  GraphicAmbientColor=[0.15 0.15 0.15 1.0]  GraphicEmissiveColor=[0.0 0.0 0.0 1.0]  GraphicShininess=75  DoExposeReferenceFrame=on  SerializedFrames=<Frames/>
  vis_pitch_hornT1 : sm_lib/Frames and Transforms/Rigid Transform  RotationMethod=RotationMatrix  FollAlignAxisA=+X  BaseAlignAxisA=+Y  FollAlignAxisB=+Y  BaseAlignAxisB=+Z  RotationStandardAxis=+Z  RotationAngle=0  RotationAngleUnits=deg  RotationArbitraryAxis=[0 0 1]  RotationSequenceAxes=FollowerAxes  RotationSequence=XYX  RotationSequenceAngles=[0 0 0]  RotationSequenceAnglesUnits=deg  RotationMatrix=[1 0 0;0 1 0;0 0 1]  Quaternion=[1 0 0 0]  TranslationMethod=Cartesian  TranslationCartesianOffset=[140 0 0]  TranslationCartesianOffsetUnits=mm  TranslationStandardAxis=+Z  TranslationStandardOffset=0  TranslationStandardOffsetUnits=m  TranslationROffset=0  TranslationROffsetUnits=m  TranslationThetaOffset=0  TranslationThetaOffsetUnits=deg  TranslationZOffset=0  TranslationZOffsetUnits=m
  vis_pitch_hornT2 : sm_lib/Frames and Transforms/Rigid Transform  RotationMethod=RotationMatrix  FollAlignAxisA=+X  BaseAlignAxisA=+Y  FollAlignAxisB=+Y  BaseAlignAxisB=+Z  RotationStandardAxis=+Z  RotationAngle=0  RotationAngleUnits=deg  RotationArbitraryAxis=[0 0 1]  RotationSequenceAxes=FollowerAxes  RotationSequence=XYX  RotationSequenceAngles=[0 0 0]  RotationSequenceAnglesUnits=deg  RotationMatrix=[1 0 0;0 1 0;0 0 1]  Quaternion=[1 0 0 0]  TranslationMethod=Cartesian  TranslationCartesianOffset=[-140 0 0]  TranslationCartesianOffsetUnits=mm  TranslationStandardAxis=+Z  TranslationStandardOffset=0  TranslationStandardOffsetUnits=m  TranslationROffset=0  TranslationROffsetUnits=m  TranslationThetaOffset=0  TranslationThetaOffsetUnits=deg  TranslationZOffset=0  TranslationZOffsetUnits=m
  vis_pitch_horn_in : nesl_utility/Simulink-PS Converter  PhysicalDomain=network_engine_domain  SubClassName=ps_input  LeftPortType=input  RightPortType=output  PseudoPeriodic=off  Frequencies=[]  NoiseDistribution=none  NoiseParameters=[]  Unit=rad  AffineConversion=off  FilteringAndDerivatives=filter  SimscapeFilterOrder=2  InputFilterTimeConstant=air_filter_s  UdotUserProvided=0
  vis_pitch_horn_q : sm_lib/Joints/Revolute Joint  JointMode=Normal  CompositeWrenchDir=FollowerOnBase  CompositeWrenchFrame=BaseFrame  SenseConstraintForce=off  SenseConstraintTorque=off  SenseTotalForce=off  SenseTotalTorque=off  PositionTargetSpecify=off  PositionTargetPriority=High  PositionTargetValue=0  PositionTargetValueUnits=deg  VelocityTargetSpecify=off  VelocityTargetPriority=High  VelocityTargetValue=0  VelocityTargetValueUnits=deg/s  EquilibriumPosition=0  EquilibriumPositionUnits=deg  SpringStiffness=0  SpringStiffnessUnits=N*m/deg  DampingCoefficient=0  DampingCoefficientUnits=N*m/(deg/s)  LowerLimitSpecify=off  LowerLimitBound=-90  LowerLimitBoundUnits=deg  LowerLimitStiffness=1e4  LowerLimitStiffnessUnits=N*m/deg  LowerLimitDamping=10  LowerLimitDampingUnits=N*m/(deg/s)  LowerLimitTransitionRegionWidth=0.1  LowerLimitTransitionRegionWidthUnits=deg  UpperLimitSpecify=off  UpperLimitBound=90  UpperLimitBoundUnits=deg  UpperLimitStiffness=1e4  UpperLimitStiffnessUnits=N*m/deg  UpperLimitDamping=10  UpperLimitDampingUnits=N*m/(deg/s)  UpperLimitTransitionRegionWidth=0.1  UpperLimitTransitionRegionWidthUnits=deg  TorqueActuationMode=ComputedTorque  MotionActuationMode=InputMotion  SensePosition=off  SenseVelocity=off  SenseAcceleration=off  SenseTorqueForce=off  SenseLowerLimitTorqueForce=off  SenseUpperLimitTorqueForce=off
  vis_pitch_horn_q_axisIn : sm_lib/Frames and Transforms/Rigid Transform  RotationMethod=RotationMatrix  FollAlignAxisA=+X  BaseAlignAxisA=+Y  FollAlignAxisB=+Y  BaseAlignAxisB=+Z  RotationStandardAxis=+Z  RotationAngle=0  RotationAngleUnits=deg  RotationArbitraryAxis=[0 0 1]  RotationSequenceAxes=FollowerAxes  RotationSequence=XYX  RotationSequenceAngles=[0 0 0]  RotationSequenceAnglesUnits=deg  RotationMatrix=[0 1 0;0 0 1;1 0 0]  Quaternion=[1 0 0 0]  TranslationMethod=Cartesian  TranslationCartesianOffset=[0 0 0]  TranslationCartesianOffsetUnits=mm  TranslationStandardAxis=+Z  TranslationStandardOffset=0  TranslationStandardOffsetUnits=m  TranslationROffset=0  TranslationROffsetUnits=m  TranslationThetaOffset=0  TranslationThetaOffsetUnits=deg  TranslationZOffset=0  TranslationZOffsetUnits=m
  vis_pitch_horn_q_axisOut : sm_lib/Frames and Transforms/Rigid Transform  RotationMethod=RotationMatrix  FollAlignAxisA=+X  BaseAlignAxisA=+Y  FollAlignAxisB=+Y  BaseAlignAxisB=+Z  RotationStandardAxis=+Z  RotationAngle=0  RotationAngleUnits=deg  RotationArbitraryAxis=[0 0 1]  RotationSequenceAxes=FollowerAxes  RotationSequence=XYX  RotationSequenceAngles=[0 0 0]  RotationSequenceAnglesUnits=deg  RotationMatrix=[0 0 1;1 0 0;0 1 0]  Quaternion=[1 0 0 0]  TranslationMethod=Cartesian  TranslationCartesianOffset=[0 0 0]  TranslationCartesianOffsetUnits=mm  TranslationStandardAxis=+Z  TranslationStandardOffset=0  TranslationStandardOffsetUnits=m  TranslationROffset=0  TranslationROffsetUnits=m  TranslationThetaOffset=0  TranslationThetaOffsetUnits=deg  TranslationZOffset=0  TranslationZOffsetUnits=m
  vis_pitch_pin : sm_lib/Body Elements/File Solid  ExtGeomFileName=/Users/ruru/Documenti-local/projects/hackathon/edth/hackathon-paris-2026/cad/stl/vis_pitch_pin.stl  UnitType=Custom  ExtGeomFileUnits=mm  StepReaderType=HEX  ExportConvexHullGeometry=off  InertiaType=CalculateFromGeometry  BasedOnType=Mass  Density=1000  DensityUnits=kg/m^3  Mass=1e-6  MassUnits=kg  CenterOfMass=[0 0 0]  CenterOfMassUnits=m  MomentsOfInertia=[1 1 1]  MomentsOfInertiaUnits=kg*m^2  ProductsOfInertia=[0 0 0]  ProductsOfInertiaUnits=kg*m^2  GraphicType=FromGeometry  MarkerShape=Sphere  MarkerSize=10  GraphicVisPropType=SimpleVisualProperties  GraphicDiffuseColor=[0.61 0.64 0.69]  GraphicOpacity=1  GraphicSpecularColor=[0.5 0.5 0.5 1.0]  GraphicAmbientColor=[0.15 0.15 0.15 1.0]  GraphicEmissiveColor=[0.0 0.0 0.0 1.0]  GraphicShininess=75  DoExposeReferenceFrame=on  SerializedFrames=<Frames/>
  vis_pitch_rod : sm_lib/Body Elements/File Solid  ExtGeomFileName=/Users/ruru/Documenti-local/projects/hackathon/edth/hackathon-paris-2026/cad/stl/vis_pitch_rod.stl  UnitType=Custom  ExtGeomFileUnits=mm  StepReaderType=HEX  ExportConvexHullGeometry=off  InertiaType=CalculateFromGeometry  BasedOnType=Mass  Density=1000  DensityUnits=kg/m^3  Mass=1e-6  MassUnits=kg  CenterOfMass=[0 0 0]  CenterOfMassUnits=m  MomentsOfInertia=[1 1 1]  MomentsOfInertiaUnits=kg*m^2  ProductsOfInertia=[0 0 0]  ProductsOfInertiaUnits=kg*m^2  GraphicType=FromGeometry  MarkerShape=Sphere  MarkerSize=10  GraphicVisPropType=SimpleVisualProperties  GraphicDiffuseColor=[0.85 0.47 0.02]  GraphicOpacity=1  GraphicSpecularColor=[0.5 0.5 0.5 1.0]  GraphicAmbientColor=[0.15 0.15 0.15 1.0]  GraphicEmissiveColor=[0.0 0.0 0.0 1.0]  GraphicShininess=75  DoExposeReferenceFrame=on  SerializedFrames=<Frames/>
  vis_pitch_rodT1 : sm_lib/Frames and Transforms/Rigid Transform  RotationMethod=RotationMatrix  FollAlignAxisA=+X  BaseAlignAxisA=+Y  FollAlignAxisB=+Y  BaseAlignAxisB=+Z  RotationStandardAxis=+Z  RotationAngle=0  RotationAngleUnits=deg  RotationArbitraryAxis=[0 0 1]  RotationSequenceAxes=FollowerAxes  RotationSequence=XYX  RotationSequenceAngles=[0 0 0]  RotationSequenceAnglesUnits=deg  RotationMatrix=[1 0 0;0 1 0;0 0 1]  Quaternion=[1 0 0 0]  TranslationMethod=Cartesian  TranslationCartesianOffset=[140 0 0]  TranslationCartesianOffsetUnits=mm  TranslationStandardAxis=+Z  TranslationStandardOffset=0  TranslationStandardOffsetUnits=m  TranslationROffset=0  TranslationROffsetUnits=m  TranslationThetaOffset=0  TranslationThetaOffsetUnits=deg  TranslationZOffset=0  TranslationZOffsetUnits=m
  vis_pitch_rodT2 : sm_lib/Frames and Transforms/Rigid Transform  RotationMethod=RotationMatrix  FollAlignAxisA=+X  BaseAlignAxisA=+Y  FollAlignAxisB=+Y  BaseAlignAxisB=+Z  RotationStandardAxis=+Z  RotationAngle=0  RotationAngleUnits=deg  RotationArbitraryAxis=[0 0 1]  RotationSequenceAxes=FollowerAxes  RotationSequence=XYX  RotationSequenceAngles=[0 0 0]  RotationSequenceAnglesUnits=deg  RotationMatrix=[1 0 0;0 1 0;0 0 1]  Quaternion=[1 0 0 0]  TranslationMethod=Cartesian  TranslationCartesianOffset=[0 0 35]  TranslationCartesianOffsetUnits=mm  TranslationStandardAxis=+Z  TranslationStandardOffset=0  TranslationStandardOffsetUnits=m  TranslationROffset=0  TranslationROffsetUnits=m  TranslationThetaOffset=0  TranslationThetaOffsetUnits=deg  TranslationZOffset=0  TranslationZOffsetUnits=m
  vis_pitch_rodT3 : sm_lib/Frames and Transforms/Rigid Transform  RotationMethod=RotationMatrix  FollAlignAxisA=+X  BaseAlignAxisA=+Y  FollAlignAxisB=+Y  BaseAlignAxisB=+Z  RotationStandardAxis=+Z  RotationAngle=0  RotationAngleUnits=deg  RotationArbitraryAxis=[0 0 1]  RotationSequenceAxes=FollowerAxes  RotationSequence=XYX  RotationSequenceAngles=[0 0 0]  RotationSequenceAnglesUnits=deg  RotationMatrix=[1 0 0;0 1 0;0 0 1]  Quaternion=[1 0 0 0]  TranslationMethod=Cartesian  TranslationCartesianOffset=[-140 0 -35]  TranslationCartesianOffsetUnits=mm  TranslationStandardAxis=+Z  TranslationStandardOffset=0  TranslationStandardOffsetUnits=m  TranslationROffset=0  TranslationROffsetUnits=m  TranslationThetaOffset=0  TranslationThetaOffsetUnits=deg  TranslationZOffset=0  TranslationZOffsetUnits=m
  vis_pitch_rod_in : nesl_utility/Simulink-PS Converter  PhysicalDomain=network_engine_domain  SubClassName=ps_input  LeftPortType=input  RightPortType=output  PseudoPeriodic=off  Frequencies=[]  NoiseDistribution=none  NoiseParameters=[]  Unit=rad  AffineConversion=off  FilteringAndDerivatives=filter  SimscapeFilterOrder=2  InputFilterTimeConstant=air_filter_s  UdotUserProvided=0
  vis_pitch_rod_inn : nesl_utility/Simulink-PS Converter  PhysicalDomain=network_engine_domain  SubClassName=ps_input  LeftPortType=input  RightPortType=output  PseudoPeriodic=off  Frequencies=[]  NoiseDistribution=none  NoiseParameters=[]  Unit=rad  AffineConversion=off  FilteringAndDerivatives=filter  SimscapeFilterOrder=2  InputFilterTimeConstant=air_filter_s  UdotUserProvided=0
  vis_pitch_rod_q : sm_lib/Joints/Revolute Joint  JointMode=Normal  CompositeWrenchDir=FollowerOnBase  CompositeWrenchFrame=BaseFrame  SenseConstraintForce=off  SenseConstraintTorque=off  SenseTotalForce=off  SenseTotalTorque=off  PositionTargetSpecify=off  PositionTargetPriority=High  PositionTargetValue=0  PositionTargetValueUnits=deg  VelocityTargetSpecify=off  VelocityTargetPriority=High  VelocityTargetValue=0  VelocityTargetValueUnits=deg/s  EquilibriumPosition=0  EquilibriumPositionUnits=deg  SpringStiffness=0  SpringStiffnessUnits=N*m/deg  DampingCoefficient=0  DampingCoefficientUnits=N*m/(deg/s)  LowerLimitSpecify=off  LowerLimitBound=-90  LowerLimitBoundUnits=deg  LowerLimitStiffness=1e4  LowerLimitStiffnessUnits=N*m/deg  LowerLimitDamping=10  LowerLimitDampingUnits=N*m/(deg/s)  LowerLimitTransitionRegionWidth=0.1  LowerLimitTransitionRegionWidthUnits=deg  UpperLimitSpecify=off  UpperLimitBound=90  UpperLimitBoundUnits=deg  UpperLimitStiffness=1e4  UpperLimitStiffnessUnits=N*m/deg  UpperLimitDamping=10  UpperLimitDampingUnits=N*m/(deg/s)  UpperLimitTransitionRegionWidth=0.1  UpperLimitTransitionRegionWidthUnits=deg  TorqueActuationMode=ComputedTorque  MotionActuationMode=InputMotion  SensePosition=off  SenseVelocity=off  SenseAcceleration=off  SenseTorqueForce=off  SenseLowerLimitTorqueForce=off  SenseUpperLimitTorqueForce=off
  vis_pitch_rod_q_axisIn : sm_lib/Frames and Transforms/Rigid Transform  RotationMethod=RotationMatrix  FollAlignAxisA=+X  BaseAlignAxisA=+Y  FollAlignAxisB=+Y  BaseAlignAxisB=+Z  RotationStandardAxis=+Z  RotationAngle=0  RotationAngleUnits=deg  RotationArbitraryAxis=[0 0 1]  RotationSequenceAxes=FollowerAxes  RotationSequence=XYX  RotationSequenceAngles=[0 0 0]  RotationSequenceAnglesUnits=deg  RotationMatrix=[0 1 0;0 0 1;1 0 0]  Quaternion=[1 0 0 0]  TranslationMethod=Cartesian  TranslationCartesianOffset=[0 0 0]  TranslationCartesianOffsetUnits=mm  TranslationStandardAxis=+Z  TranslationStandardOffset=0  TranslationStandardOffsetUnits=m  TranslationROffset=0  TranslationROffsetUnits=m  TranslationThetaOffset=0  TranslationThetaOffsetUnits=deg  TranslationZOffset=0  TranslationZOffsetUnits=m
  vis_pitch_rod_q_axisOut : sm_lib/Frames and Transforms/Rigid Transform  RotationMethod=RotationMatrix  FollAlignAxisA=+X  BaseAlignAxisA=+Y  FollAlignAxisB=+Y  BaseAlignAxisB=+Z  RotationStandardAxis=+Z  RotationAngle=0  RotationAngleUnits=deg  RotationArbitraryAxis=[0 0 1]  RotationSequenceAxes=FollowerAxes  RotationSequence=XYX  RotationSequenceAngles=[0 0 0]  RotationSequenceAnglesUnits=deg  RotationMatrix=[0 0 1;1 0 0;0 1 0]  Quaternion=[1 0 0 0]  TranslationMethod=Cartesian  TranslationCartesianOffset=[0 0 0]  TranslationCartesianOffsetUnits=mm  TranslationStandardAxis=+Z  TranslationStandardOffset=0  TranslationStandardOffsetUnits=m  TranslationROffset=0  TranslationROffsetUnits=m  TranslationThetaOffset=0  TranslationThetaOffsetUnits=deg  TranslationZOffset=0  TranslationZOffsetUnits=m
  vis_pitch_rod_qn : sm_lib/Joints/Revolute Joint  JointMode=Normal  CompositeWrenchDir=FollowerOnBase  CompositeWrenchFrame=BaseFrame  SenseConstraintForce=off  SenseConstraintTorque=off  SenseTotalForce=off  SenseTotalTorque=off  PositionTargetSpecify=off  PositionTargetPriority=High  PositionTargetValue=0  PositionTargetValueUnits=deg  VelocityTargetSpecify=off  VelocityTargetPriority=High  VelocityTargetValue=0  VelocityTargetValueUnits=deg/s  EquilibriumPosition=0  EquilibriumPositionUnits=deg  SpringStiffness=0  SpringStiffnessUnits=N*m/deg  DampingCoefficient=0  DampingCoefficientUnits=N*m/(deg/s)  LowerLimitSpecify=off  LowerLimitBound=-90  LowerLimitBoundUnits=deg  LowerLimitStiffness=1e4  LowerLimitStiffnessUnits=N*m/deg  LowerLimitDamping=10  LowerLimitDampingUnits=N*m/(deg/s)  LowerLimitTransitionRegionWidth=0.1  LowerLimitTransitionRegionWidthUnits=deg  UpperLimitSpecify=off  UpperLimitBound=90  UpperLimitBoundUnits=deg  UpperLimitStiffness=1e4  UpperLimitStiffnessUnits=N*m/deg  UpperLimitDamping=10  UpperLimitDampingUnits=N*m/(deg/s)  UpperLimitTransitionRegionWidth=0.1  UpperLimitTransitionRegionWidthUnits=deg  TorqueActuationMode=ComputedTorque  MotionActuationMode=InputMotion  SensePosition=off  SenseVelocity=off  SenseAcceleration=off  SenseTorqueForce=off  SenseLowerLimitTorqueForce=off  SenseUpperLimitTorqueForce=off
  vis_pitch_rod_qn_axisIn : sm_lib/Frames and Transforms/Rigid Transform  RotationMethod=RotationMatrix  FollAlignAxisA=+X  BaseAlignAxisA=+Y  FollAlignAxisB=+Y  BaseAlignAxisB=+Z  RotationStandardAxis=+Z  RotationAngle=0  RotationAngleUnits=deg  RotationArbitraryAxis=[0 0 1]  RotationSequenceAxes=FollowerAxes  RotationSequence=XYX  RotationSequenceAngles=[0 0 0]  RotationSequenceAnglesUnits=deg  RotationMatrix=[0 1 0;0 0 1;1 0 0]  Quaternion=[1 0 0 0]  TranslationMethod=Cartesian  TranslationCartesianOffset=[0 0 0]  TranslationCartesianOffsetUnits=mm  TranslationStandardAxis=+Z  TranslationStandardOffset=0  TranslationStandardOffsetUnits=m  TranslationROffset=0  TranslationROffsetUnits=m  TranslationThetaOffset=0  TranslationThetaOffsetUnits=deg  TranslationZOffset=0  TranslationZOffsetUnits=m
  vis_pitch_rod_qn_axisOut : sm_lib/Frames and Transforms/Rigid Transform  RotationMethod=RotationMatrix  FollAlignAxisA=+X  BaseAlignAxisA=+Y  FollAlignAxisB=+Y  BaseAlignAxisB=+Z  RotationStandardAxis=+Z  RotationAngle=0  RotationAngleUnits=deg  RotationArbitraryAxis=[0 0 1]  RotationSequenceAxes=FollowerAxes  RotationSequence=XYX  RotationSequenceAngles=[0 0 0]  RotationSequenceAnglesUnits=deg  RotationMatrix=[0 0 1;1 0 0;0 1 0]  Quaternion=[1 0 0 0]  TranslationMethod=Cartesian  TranslationCartesianOffset=[0 0 0]  TranslationCartesianOffsetUnits=mm  TranslationStandardAxis=+Z  TranslationStandardOffset=0  TranslationStandardOffsetUnits=m  TranslationROffset=0  TranslationROffsetUnits=m  TranslationThetaOffset=0  TranslationThetaOffsetUnits=deg  TranslationZOffset=0  TranslationZOffsetUnits=m
  vis_pitch_servo_horn : sm_lib/Body Elements/File Solid  ExtGeomFileName=/Users/ruru/Documenti-local/projects/hackathon/edth/hackathon-paris-2026/cad/stl/vis_pitch_servo_horn.stl  UnitType=Custom  ExtGeomFileUnits=mm  StepReaderType=HEX  ExportConvexHullGeometry=off  InertiaType=CalculateFromGeometry  BasedOnType=Mass  Density=1000  DensityUnits=kg/m^3  Mass=1e-6  MassUnits=kg  CenterOfMass=[0 0 0]  CenterOfMassUnits=m  MomentsOfInertia=[1 1 1]  MomentsOfInertiaUnits=kg*m^2  ProductsOfInertia=[0 0 0]  ProductsOfInertiaUnits=kg*m^2  GraphicType=FromGeometry  MarkerShape=Sphere  MarkerSize=10  GraphicVisPropType=SimpleVisualProperties  GraphicDiffuseColor=[0.85 0.47 0.02]  GraphicOpacity=1  GraphicSpecularColor=[0.5 0.5 0.5 1.0]  GraphicAmbientColor=[0.15 0.15 0.15 1.0]  GraphicEmissiveColor=[0.0 0.0 0.0 1.0]  GraphicShininess=75  DoExposeReferenceFrame=on  SerializedFrames=<Frames/>
  vis_pitch_shafts : sm_lib/Body Elements/File Solid  ExtGeomFileName=/Users/ruru/Documenti-local/projects/hackathon/edth/hackathon-paris-2026/cad/stl/vis_pitch_shafts.stl  UnitType=Custom  ExtGeomFileUnits=mm  StepReaderType=HEX  ExportConvexHullGeometry=off  InertiaType=CalculateFromGeometry  BasedOnType=Mass  Density=1000  DensityUnits=kg/m^3  Mass=1e-6  MassUnits=kg  CenterOfMass=[0 0 0]  CenterOfMassUnits=m  MomentsOfInertia=[1 1 1]  MomentsOfInertiaUnits=kg*m^2  ProductsOfInertia=[0 0 0]  ProductsOfInertiaUnits=kg*m^2  GraphicType=FromGeometry  MarkerShape=Sphere  MarkerSize=10  GraphicVisPropType=SimpleVisualProperties  GraphicDiffuseColor=[0.61 0.64 0.69]  GraphicOpacity=1  GraphicSpecularColor=[0.5 0.5 0.5 1.0]  GraphicAmbientColor=[0.15 0.15 0.15 1.0]  GraphicEmissiveColor=[0.0 0.0 0.0 1.0]  GraphicShininess=75  DoExposeReferenceFrame=on  SerializedFrames=<Frames/>
  vis_roll_hornT1 : sm_lib/Frames and Transforms/Rigid Transform  RotationMethod=RotationMatrix  FollAlignAxisA=+X  BaseAlignAxisA=+Y  FollAlignAxisB=+Y  BaseAlignAxisB=+Z  RotationStandardAxis=+Z  RotationAngle=0  RotationAngleUnits=deg  RotationArbitraryAxis=[0 0 1]  RotationSequenceAxes=FollowerAxes  RotationSequence=XYX  RotationSequenceAngles=[0 0 0]  RotationSequenceAnglesUnits=deg  RotationMatrix=[1 0 0;0 1 0;0 0 1]  Quaternion=[1 0 0 0]  TranslationMethod=Cartesian  TranslationCartesianOffset=[0 0 -127]  TranslationCartesianOffsetUnits=mm  TranslationStandardAxis=+Z  TranslationStandardOffset=0  TranslationStandardOffsetUnits=m  TranslationROffset=0  TranslationROffsetUnits=m  TranslationThetaOffset=0  TranslationThetaOffsetUnits=deg  TranslationZOffset=0  TranslationZOffsetUnits=m
  vis_roll_hornT2 : sm_lib/Frames and Transforms/Rigid Transform  RotationMethod=RotationMatrix  FollAlignAxisA=+X  BaseAlignAxisA=+Y  FollAlignAxisB=+Y  BaseAlignAxisB=+Z  RotationStandardAxis=+Z  RotationAngle=0  RotationAngleUnits=deg  RotationArbitraryAxis=[0 0 1]  RotationSequenceAxes=FollowerAxes  RotationSequence=XYX  RotationSequenceAngles=[0 0 0]  RotationSequenceAnglesUnits=deg  RotationMatrix=[1 0 0;0 1 0;0 0 1]  Quaternion=[1 0 0 0]  TranslationMethod=Cartesian  TranslationCartesianOffset=[0 0 127]  TranslationCartesianOffsetUnits=mm  TranslationStandardAxis=+Z  TranslationStandardOffset=0  TranslationStandardOffsetUnits=m  TranslationROffset=0  TranslationROffsetUnits=m  TranslationThetaOffset=0  TranslationThetaOffsetUnits=deg  TranslationZOffset=0  TranslationZOffsetUnits=m
  vis_roll_horn_in : nesl_utility/Simulink-PS Converter  PhysicalDomain=network_engine_domain  SubClassName=ps_input  LeftPortType=input  RightPortType=output  PseudoPeriodic=off  Frequencies=[]  NoiseDistribution=none  NoiseParameters=[]  Unit=rad  AffineConversion=off  FilteringAndDerivatives=filter  SimscapeFilterOrder=2  InputFilterTimeConstant=air_filter_s  UdotUserProvided=0
  vis_roll_horn_q : sm_lib/Joints/Revolute Joint  JointMode=Normal  CompositeWrenchDir=FollowerOnBase  CompositeWrenchFrame=BaseFrame  SenseConstraintForce=off  SenseConstraintTorque=off  SenseTotalForce=off  SenseTotalTorque=off  PositionTargetSpecify=off  PositionTargetPriority=High  PositionTargetValue=0  PositionTargetValueUnits=deg  VelocityTargetSpecify=off  VelocityTargetPriority=High  VelocityTargetValue=0  VelocityTargetValueUnits=deg/s  EquilibriumPosition=0  EquilibriumPositionUnits=deg  SpringStiffness=0  SpringStiffnessUnits=N*m/deg  DampingCoefficient=0  DampingCoefficientUnits=N*m/(deg/s)  LowerLimitSpecify=off  LowerLimitBound=-90  LowerLimitBoundUnits=deg  LowerLimitStiffness=1e4  LowerLimitStiffnessUnits=N*m/deg  LowerLimitDamping=10  LowerLimitDampingUnits=N*m/(deg/s)  LowerLimitTransitionRegionWidth=0.1  LowerLimitTransitionRegionWidthUnits=deg  UpperLimitSpecify=off  UpperLimitBound=90  UpperLimitBoundUnits=deg  UpperLimitStiffness=1e4  UpperLimitStiffnessUnits=N*m/deg  UpperLimitDamping=10  UpperLimitDampingUnits=N*m/(deg/s)  UpperLimitTransitionRegionWidth=0.1  UpperLimitTransitionRegionWidthUnits=deg  TorqueActuationMode=ComputedTorque  MotionActuationMode=InputMotion  SensePosition=off  SenseVelocity=off  SenseAcceleration=off  SenseTorqueForce=off  SenseLowerLimitTorqueForce=off  SenseUpperLimitTorqueForce=off
  vis_roll_horn_q_axisIn : sm_lib/Frames and Transforms/Rigid Transform  RotationMethod=RotationMatrix  FollAlignAxisA=+X  BaseAlignAxisA=+Y  FollAlignAxisB=+Y  BaseAlignAxisB=+Z  RotationStandardAxis=+Z  RotationAngle=0  RotationAngleUnits=deg  RotationArbitraryAxis=[0 0 1]  RotationSequenceAxes=FollowerAxes  RotationSequence=XYX  RotationSequenceAngles=[0 0 0]  RotationSequenceAnglesUnits=deg  RotationMatrix=[0 0 1;1 0 0;0 1 0]  Quaternion=[1 0 0 0]  TranslationMethod=Cartesian  TranslationCartesianOffset=[0 0 0]  TranslationCartesianOffsetUnits=mm  TranslationStandardAxis=+Z  TranslationStandardOffset=0  TranslationStandardOffsetUnits=m  TranslationROffset=0  TranslationROffsetUnits=m  TranslationThetaOffset=0  TranslationThetaOffsetUnits=deg  TranslationZOffset=0  TranslationZOffsetUnits=m
  vis_roll_horn_q_axisOut : sm_lib/Frames and Transforms/Rigid Transform  RotationMethod=RotationMatrix  FollAlignAxisA=+X  BaseAlignAxisA=+Y  FollAlignAxisB=+Y  BaseAlignAxisB=+Z  RotationStandardAxis=+Z  RotationAngle=0  RotationAngleUnits=deg  RotationArbitraryAxis=[0 0 1]  RotationSequenceAxes=FollowerAxes  RotationSequence=XYX  RotationSequenceAngles=[0 0 0]  RotationSequenceAnglesUnits=deg  RotationMatrix=[0 1 0;0 0 1;1 0 0]  Quaternion=[1 0 0 0]  TranslationMethod=Cartesian  TranslationCartesianOffset=[0 0 0]  TranslationCartesianOffsetUnits=mm  TranslationStandardAxis=+Z  TranslationStandardOffset=0  TranslationStandardOffsetUnits=m  TranslationROffset=0  TranslationROffsetUnits=m  TranslationThetaOffset=0  TranslationThetaOffsetUnits=deg  TranslationZOffset=0  TranslationZOffsetUnits=m
  vis_roll_pin : sm_lib/Body Elements/File Solid  ExtGeomFileName=/Users/ruru/Documenti-local/projects/hackathon/edth/hackathon-paris-2026/cad/stl/vis_roll_pin.stl  UnitType=Custom  ExtGeomFileUnits=mm  StepReaderType=HEX  ExportConvexHullGeometry=off  InertiaType=CalculateFromGeometry  BasedOnType=Mass  Density=1000  DensityUnits=kg/m^3  Mass=1e-6  MassUnits=kg  CenterOfMass=[0 0 0]  CenterOfMassUnits=m  MomentsOfInertia=[1 1 1]  MomentsOfInertiaUnits=kg*m^2  ProductsOfInertia=[0 0 0]  ProductsOfInertiaUnits=kg*m^2  GraphicType=FromGeometry  MarkerShape=Sphere  MarkerSize=10  GraphicVisPropType=SimpleVisualProperties  GraphicDiffuseColor=[0.61 0.64 0.69]  GraphicOpacity=1  GraphicSpecularColor=[0.5 0.5 0.5 1.0]  GraphicAmbientColor=[0.15 0.15 0.15 1.0]  GraphicEmissiveColor=[0.0 0.0 0.0 1.0]  GraphicShininess=75  DoExposeReferenceFrame=on  SerializedFrames=<Frames/>
  vis_roll_rod : sm_lib/Body Elements/File Solid  ExtGeomFileName=/Users/ruru/Documenti-local/projects/hackathon/edth/hackathon-paris-2026/cad/stl/vis_roll_rod.stl  UnitType=Custom  ExtGeomFileUnits=mm  StepReaderType=HEX  ExportConvexHullGeometry=off  InertiaType=CalculateFromGeometry  BasedOnType=Mass  Density=1000  DensityUnits=kg/m^3  Mass=1e-6  MassUnits=kg  CenterOfMass=[0 0 0]  CenterOfMassUnits=m  MomentsOfInertia=[1 1 1]  MomentsOfInertiaUnits=kg*m^2  ProductsOfInertia=[0 0 0]  ProductsOfInertiaUnits=kg*m^2  GraphicType=FromGeometry  MarkerShape=Sphere  MarkerSize=10  GraphicVisPropType=SimpleVisualProperties  GraphicDiffuseColor=[0.85 0.47 0.02]  GraphicOpacity=1  GraphicSpecularColor=[0.5 0.5 0.5 1.0]  GraphicAmbientColor=[0.15 0.15 0.15 1.0]  GraphicEmissiveColor=[0.0 0.0 0.0 1.0]  GraphicShininess=75  DoExposeReferenceFrame=on  SerializedFrames=<Frames/>
  vis_roll_rodT1 : sm_lib/Frames and Transforms/Rigid Transform  RotationMethod=RotationMatrix  FollAlignAxisA=+X  BaseAlignAxisA=+Y  FollAlignAxisB=+Y  BaseAlignAxisB=+Z  RotationStandardAxis=+Z  RotationAngle=0  RotationAngleUnits=deg  RotationArbitraryAxis=[0 0 1]  RotationSequenceAxes=FollowerAxes  RotationSequence=XYX  RotationSequenceAngles=[0 0 0]  RotationSequenceAnglesUnits=deg  RotationMatrix=[1 0 0;0 1 0;0 0 1]  Quaternion=[1 0 0 0]  TranslationMethod=Cartesian  TranslationCartesianOffset=[0 0 -127]  TranslationCartesianOffsetUnits=mm  TranslationStandardAxis=+Z  TranslationStandardOffset=0  TranslationStandardOffsetUnits=m  TranslationROffset=0  TranslationROffsetUnits=m  TranslationThetaOffset=0  TranslationThetaOffsetUnits=deg  TranslationZOffset=0  TranslationZOffsetUnits=m
  vis_roll_rodT2 : sm_lib/Frames and Transforms/Rigid Transform  RotationMethod=RotationMatrix  FollAlignAxisA=+X  BaseAlignAxisA=+Y  FollAlignAxisB=+Y  BaseAlignAxisB=+Z  RotationStandardAxis=+Z  RotationAngle=0  RotationAngleUnits=deg  RotationArbitraryAxis=[0 0 1]  RotationSequenceAxes=FollowerAxes  RotationSequence=XYX  RotationSequenceAngles=[0 0 0]  RotationSequenceAnglesUnits=deg  RotationMatrix=[1 0 0;0 1 0;0 0 1]  Quaternion=[1 0 0 0]  TranslationMethod=Cartesian  TranslationCartesianOffset=[0 25 0]  TranslationCartesianOffsetUnits=mm  TranslationStandardAxis=+Z  TranslationStandardOffset=0  TranslationStandardOffsetUnits=m  TranslationROffset=0  TranslationROffsetUnits=m  TranslationThetaOffset=0  TranslationThetaOffsetUnits=deg  TranslationZOffset=0  TranslationZOffsetUnits=m
  vis_roll_rodT3 : sm_lib/Frames and Transforms/Rigid Transform  RotationMethod=RotationMatrix  FollAlignAxisA=+X  BaseAlignAxisA=+Y  FollAlignAxisB=+Y  BaseAlignAxisB=+Z  RotationStandardAxis=+Z  RotationAngle=0  RotationAngleUnits=deg  RotationArbitraryAxis=[0 0 1]  RotationSequenceAxes=FollowerAxes  RotationSequence=XYX  RotationSequenceAngles=[0 0 0]  RotationSequenceAnglesUnits=deg  RotationMatrix=[1 0 0;0 1 0;0 0 1]  Quaternion=[1 0 0 0]  TranslationMethod=Cartesian  TranslationCartesianOffset=[0 -25 127]  TranslationCartesianOffsetUnits=mm  TranslationStandardAxis=+Z  TranslationStandardOffset=0  TranslationStandardOffsetUnits=m  TranslationROffset=0  TranslationROffsetUnits=m  TranslationThetaOffset=0  TranslationThetaOffsetUnits=deg  TranslationZOffset=0  TranslationZOffsetUnits=m
  vis_roll_rod_in : nesl_utility/Simulink-PS Converter  PhysicalDomain=network_engine_domain  SubClassName=ps_input  LeftPortType=input  RightPortType=output  PseudoPeriodic=off  Frequencies=[]  NoiseDistribution=none  NoiseParameters=[]  Unit=rad  AffineConversion=off  FilteringAndDerivatives=filter  SimscapeFilterOrder=2  InputFilterTimeConstant=air_filter_s  UdotUserProvided=0
  vis_roll_rod_inn : nesl_utility/Simulink-PS Converter  PhysicalDomain=network_engine_domain  SubClassName=ps_input  LeftPortType=input  RightPortType=output  PseudoPeriodic=off  Frequencies=[]  NoiseDistribution=none  NoiseParameters=[]  Unit=rad  AffineConversion=off  FilteringAndDerivatives=filter  SimscapeFilterOrder=2  InputFilterTimeConstant=air_filter_s  UdotUserProvided=0
  vis_roll_rod_q : sm_lib/Joints/Revolute Joint  JointMode=Normal  CompositeWrenchDir=FollowerOnBase  CompositeWrenchFrame=BaseFrame  SenseConstraintForce=off  SenseConstraintTorque=off  SenseTotalForce=off  SenseTotalTorque=off  PositionTargetSpecify=off  PositionTargetPriority=High  PositionTargetValue=0  PositionTargetValueUnits=deg  VelocityTargetSpecify=off  VelocityTargetPriority=High  VelocityTargetValue=0  VelocityTargetValueUnits=deg/s  EquilibriumPosition=0  EquilibriumPositionUnits=deg  SpringStiffness=0  SpringStiffnessUnits=N*m/deg  DampingCoefficient=0  DampingCoefficientUnits=N*m/(deg/s)  LowerLimitSpecify=off  LowerLimitBound=-90  LowerLimitBoundUnits=deg  LowerLimitStiffness=1e4  LowerLimitStiffnessUnits=N*m/deg  LowerLimitDamping=10  LowerLimitDampingUnits=N*m/(deg/s)  LowerLimitTransitionRegionWidth=0.1  LowerLimitTransitionRegionWidthUnits=deg  UpperLimitSpecify=off  UpperLimitBound=90  UpperLimitBoundUnits=deg  UpperLimitStiffness=1e4  UpperLimitStiffnessUnits=N*m/deg  UpperLimitDamping=10  UpperLimitDampingUnits=N*m/(deg/s)  UpperLimitTransitionRegionWidth=0.1  UpperLimitTransitionRegionWidthUnits=deg  TorqueActuationMode=ComputedTorque  MotionActuationMode=InputMotion  SensePosition=off  SenseVelocity=off  SenseAcceleration=off  SenseTorqueForce=off  SenseLowerLimitTorqueForce=off  SenseUpperLimitTorqueForce=off
  vis_roll_rod_q_axisIn : sm_lib/Frames and Transforms/Rigid Transform  RotationMethod=RotationMatrix  FollAlignAxisA=+X  BaseAlignAxisA=+Y  FollAlignAxisB=+Y  BaseAlignAxisB=+Z  RotationStandardAxis=+Z  RotationAngle=0  RotationAngleUnits=deg  RotationArbitraryAxis=[0 0 1]  RotationSequenceAxes=FollowerAxes  RotationSequence=XYX  RotationSequenceAngles=[0 0 0]  RotationSequenceAnglesUnits=deg  RotationMatrix=[0 0 1;1 0 0;0 1 0]  Quaternion=[1 0 0 0]  TranslationMethod=Cartesian  TranslationCartesianOffset=[0 0 0]  TranslationCartesianOffsetUnits=mm  TranslationStandardAxis=+Z  TranslationStandardOffset=0  TranslationStandardOffsetUnits=m  TranslationROffset=0  TranslationROffsetUnits=m  TranslationThetaOffset=0  TranslationThetaOffsetUnits=deg  TranslationZOffset=0  TranslationZOffsetUnits=m
  vis_roll_rod_q_axisOut : sm_lib/Frames and Transforms/Rigid Transform  RotationMethod=RotationMatrix  FollAlignAxisA=+X  BaseAlignAxisA=+Y  FollAlignAxisB=+Y  BaseAlignAxisB=+Z  RotationStandardAxis=+Z  RotationAngle=0  RotationAngleUnits=deg  RotationArbitraryAxis=[0 0 1]  RotationSequenceAxes=FollowerAxes  RotationSequence=XYX  RotationSequenceAngles=[0 0 0]  RotationSequenceAnglesUnits=deg  RotationMatrix=[0 1 0;0 0 1;1 0 0]  Quaternion=[1 0 0 0]  TranslationMethod=Cartesian  TranslationCartesianOffset=[0 0 0]  TranslationCartesianOffsetUnits=mm  TranslationStandardAxis=+Z  TranslationStandardOffset=0  TranslationStandardOffsetUnits=m  TranslationROffset=0  TranslationROffsetUnits=m  TranslationThetaOffset=0  TranslationThetaOffsetUnits=deg  TranslationZOffset=0  TranslationZOffsetUnits=m
  vis_roll_rod_qn : sm_lib/Joints/Revolute Joint  JointMode=Normal  CompositeWrenchDir=FollowerOnBase  CompositeWrenchFrame=BaseFrame  SenseConstraintForce=off  SenseConstraintTorque=off  SenseTotalForce=off  SenseTotalTorque=off  PositionTargetSpecify=off  PositionTargetPriority=High  PositionTargetValue=0  PositionTargetValueUnits=deg  VelocityTargetSpecify=off  VelocityTargetPriority=High  VelocityTargetValue=0  VelocityTargetValueUnits=deg/s  EquilibriumPosition=0  EquilibriumPositionUnits=deg  SpringStiffness=0  SpringStiffnessUnits=N*m/deg  DampingCoefficient=0  DampingCoefficientUnits=N*m/(deg/s)  LowerLimitSpecify=off  LowerLimitBound=-90  LowerLimitBoundUnits=deg  LowerLimitStiffness=1e4  LowerLimitStiffnessUnits=N*m/deg  LowerLimitDamping=10  LowerLimitDampingUnits=N*m/(deg/s)  LowerLimitTransitionRegionWidth=0.1  LowerLimitTransitionRegionWidthUnits=deg  UpperLimitSpecify=off  UpperLimitBound=90  UpperLimitBoundUnits=deg  UpperLimitStiffness=1e4  UpperLimitStiffnessUnits=N*m/deg  UpperLimitDamping=10  UpperLimitDampingUnits=N*m/(deg/s)  UpperLimitTransitionRegionWidth=0.1  UpperLimitTransitionRegionWidthUnits=deg  TorqueActuationMode=ComputedTorque  MotionActuationMode=InputMotion  SensePosition=off  SenseVelocity=off  SenseAcceleration=off  SenseTorqueForce=off  SenseLowerLimitTorqueForce=off  SenseUpperLimitTorqueForce=off
  vis_roll_rod_qn_axisIn : sm_lib/Frames and Transforms/Rigid Transform  RotationMethod=RotationMatrix  FollAlignAxisA=+X  BaseAlignAxisA=+Y  FollAlignAxisB=+Y  BaseAlignAxisB=+Z  RotationStandardAxis=+Z  RotationAngle=0  RotationAngleUnits=deg  RotationArbitraryAxis=[0 0 1]  RotationSequenceAxes=FollowerAxes  RotationSequence=XYX  RotationSequenceAngles=[0 0 0]  RotationSequenceAnglesUnits=deg  RotationMatrix=[0 0 1;1 0 0;0 1 0]  Quaternion=[1 0 0 0]  TranslationMethod=Cartesian  TranslationCartesianOffset=[0 0 0]  TranslationCartesianOffsetUnits=mm  TranslationStandardAxis=+Z  TranslationStandardOffset=0  TranslationStandardOffsetUnits=m  TranslationROffset=0  TranslationROffsetUnits=m  TranslationThetaOffset=0  TranslationThetaOffsetUnits=deg  TranslationZOffset=0  TranslationZOffsetUnits=m
  vis_roll_rod_qn_axisOut : sm_lib/Frames and Transforms/Rigid Transform  RotationMethod=RotationMatrix  FollAlignAxisA=+X  BaseAlignAxisA=+Y  FollAlignAxisB=+Y  BaseAlignAxisB=+Z  RotationStandardAxis=+Z  RotationAngle=0  RotationAngleUnits=deg  RotationArbitraryAxis=[0 0 1]  RotationSequenceAxes=FollowerAxes  RotationSequence=XYX  RotationSequenceAngles=[0 0 0]  RotationSequenceAnglesUnits=deg  RotationMatrix=[0 1 0;0 0 1;1 0 0]  Quaternion=[1 0 0 0]  TranslationMethod=Cartesian  TranslationCartesianOffset=[0 0 0]  TranslationCartesianOffsetUnits=mm  TranslationStandardAxis=+Z  TranslationStandardOffset=0  TranslationStandardOffsetUnits=m  TranslationROffset=0  TranslationROffsetUnits=m  TranslationThetaOffset=0  TranslationThetaOffsetUnits=deg  TranslationZOffset=0  TranslationZOffsetUnits=m
  vis_roll_servo_horn : sm_lib/Body Elements/File Solid  ExtGeomFileName=/Users/ruru/Documenti-local/projects/hackathon/edth/hackathon-paris-2026/cad/stl/vis_roll_servo_horn.stl  UnitType=Custom  ExtGeomFileUnits=mm  StepReaderType=HEX  ExportConvexHullGeometry=off  InertiaType=CalculateFromGeometry  BasedOnType=Mass  Density=1000  DensityUnits=kg/m^3  Mass=1e-6  MassUnits=kg  CenterOfMass=[0 0 0]  CenterOfMassUnits=m  MomentsOfInertia=[1 1 1]  MomentsOfInertiaUnits=kg*m^2  ProductsOfInertia=[0 0 0]  ProductsOfInertiaUnits=kg*m^2  GraphicType=FromGeometry  MarkerShape=Sphere  MarkerSize=10  GraphicVisPropType=SimpleVisualProperties  GraphicDiffuseColor=[0.85 0.47 0.02]  GraphicOpacity=1  GraphicSpecularColor=[0.5 0.5 0.5 1.0]  GraphicAmbientColor=[0.15 0.15 0.15 1.0]  GraphicEmissiveColor=[0.0 0.0 0.0 1.0]  GraphicShininess=75  DoExposeReferenceFrame=on  SerializedFrames=<Frames/>
  vis_roll_shafts : sm_lib/Body Elements/File Solid  ExtGeomFileName=/Users/ruru/Documenti-local/projects/hackathon/edth/hackathon-paris-2026/cad/stl/vis_roll_shafts.stl  UnitType=Custom  ExtGeomFileUnits=mm  StepReaderType=HEX  ExportConvexHullGeometry=off  InertiaType=CalculateFromGeometry  BasedOnType=Mass  Density=1000  DensityUnits=kg/m^3  Mass=1e-6  MassUnits=kg  CenterOfMass=[0 0 0]  CenterOfMassUnits=m  MomentsOfInertia=[1 1 1]  MomentsOfInertiaUnits=kg*m^2  ProductsOfInertia=[0 0 0]  ProductsOfInertiaUnits=kg*m^2  GraphicType=FromGeometry  MarkerShape=Sphere  MarkerSize=10  GraphicVisPropType=SimpleVisualProperties  GraphicDiffuseColor=[0.61 0.64 0.69]  GraphicOpacity=1  GraphicSpecularColor=[0.5 0.5 0.5 1.0]  GraphicAmbientColor=[0.15 0.15 0.15 1.0]  GraphicEmissiveColor=[0.0 0.0 0.0 1.0]  GraphicShininess=75  DoExposeReferenceFrame=on  SerializedFrames=<Frames/>
  wires:
  R_ps/1 -> antenna_angles/1(R)
  clock/1 -> udp_live_in/1
  air_in/1 -> source/1
  udp_live_in/1 -> source/2
  source/1 -> air_demux/1
  air_demux/1 -> air_roll_in/1, air_mux/1
  air_demux/2 -> air_pitch_in/1, air_mux/2
  air_demux/3 -> air_yaw_in/1, air_mux/3
  air_demux/6 -> gravity_in/1
  air_demux/4 -> lead/1
  air_demux/5 -> cmd_sum/1
  lead/1 -> cmd_sum/2
  cmd_sum/1 -> dead_time/1
  dead_time/1 -> mount_task/1
  mount_task/1 -> travel_limit/1
  travel_limit/1 -> pwm_frame/1
  pwm_frame/1 -> servo/1(cmd), cmd_deg/1
  SV/1 -> servo/6(SV)
  servo/2(qmdd) -> motor_rate/1
  motor_rate/1 -> motor_angle/1, servo/5(qmd)
  motor_angle/1 -> servo/4(qm)
  q_1/1 -> q_mux/1
  q_2/1 -> q_mux/2
  qd_1/1 -> qd_mux/1
  qd_2/1 -> qd_mux/2
  q_mux/1 -> servo/2(q), q_vis_delay/1, q_deg/1
  qd_mux/1 -> servo/3(qd)
  servo/1(tgear) -> tau_demux/1, log_mux/4
  tau_demux/1 -> torque_in1/1
  tau_demux/2 -> torque_in2/1
  q_vis_delay/1 -> q_vis/1, q_vis_neg/1
  q_vis_neg/1 -> q_vis_n/1
  q_vis/1 -> vis_roll_horn_in/1, vis_roll_rod_in/1
  q_vis_n/1 -> vis_roll_rod_inn/1
  q_vis/2 -> vis_pitch_horn_in/1, vis_pitch_rod_in/1
  q_vis_n/2 -> vis_pitch_rod_inn/1
  air_mux/1 -> air_deg/1
  air_deg/1 -> log_mux/1
  antenna_angles/1(ant) -> log_mux/2
  q_deg/1 -> log_mux/3
  servo/3(sat) -> log_mux/5
  cmd_deg/1 -> log_mux/6
  log_mux/1 -> log/1, live_view/1
  connections:
  Mechanism Configuration/RConn1 -- World/RConn1 -- Solver Configuration/RConn1 -- air_yaw_axisIn/LConn1 -- antenna_attitude/LConn1
  air_yaw_axisIn/RConn1 -- air_yaw/LConn1
  air_yaw/RConn1 -- air_yaw_axisOut/LConn1
  air_pitch_axisIn/RConn1 -- air_pitch/LConn1
  air_pitch/RConn1 -- air_pitch_axisOut/LConn1
  air_roll_axisIn/RConn1 -- air_roll/LConn1
  air_roll/RConn1 -- air_roll_axisOut/LConn1
  air_yaw_axisOut/RConn1 -- air_pitch_axisIn/LConn1
  air_pitch_axisOut/RConn1 -- air_roll_axisIn/LConn1
  airframe_deck_T/LConn1 -- air_roll_axisOut/RConn1 -- post_servo_side/RConn1 -- post_bearing_side/RConn1 -- roll_servo_T/LConn1 -- gimbal_roll_axisIn/LConn1 -- vis_cable/RConn1 -- vis_roll_hornT1/LConn1 -- vis_roll_rodT1/LConn1
  airframe_deck_T/RConn1 -- airframe_deck/RConn1
  roll_servo_T/RConn1 -- roll_servo/RConn1
  gimbal_roll_axisIn/RConn1 -- gimbal_roll/LConn1
  gimbal_roll/RConn1 -- gimbal_roll_axisOut/LConn1
  roll_frame/RConn1 -- gimbal_roll_axisOut/RConn1 -- pitch_servo_T/LConn1 -- gimbal_pitch_axisIn/LConn1 -- vis_roll_shafts/RConn1 -- vis_roll_pin/RConn1 -- vis_pitch_hornT1/LConn1 -- vis_pitch_rodT1/LConn1
  pitch_servo_T/RConn1 -- pitch_servo/RConn1
  gimbal_pitch_axisIn/RConn1 -- gimbal_pitch/LConn1
  gimbal_pitch/RConn1 -- gimbal_pitch_axisOut/LConn1
  antenna_brackets/RConn1 -- gimbal_pitch_axisOut/RConn1 -- antenna_cog_T/LConn1 -- antenna_attitude/RConn1 -- vis_pitch_shafts/RConn1 -- vis_pitch_pin/RConn1
  antenna_cog_T/RConn1 -- antenna/RConn1
  antenna_attitude/RConn2 -- R_ps/LConn1
  air_roll_in/RConn1 -- air_roll/LConn2
  air_pitch_in/RConn1 -- air_pitch/LConn2
  air_yaw_in/RConn1 -- air_yaw/LConn2
  gravity_in/RConn1 -- Mechanism Configuration/LConn1
  gimbal_roll/RConn2 -- q_1/LConn1
  gimbal_pitch/RConn2 -- q_2/LConn1
  gimbal_roll/RConn3 -- qd_1/LConn1
  gimbal_pitch/RConn3 -- qd_2/LConn1
  torque_in1/RConn1 -- gimbal_roll/LConn2
  torque_in2/RConn1 -- gimbal_pitch/LConn2
  vis_roll_horn_q_axisIn/RConn1 -- vis_roll_horn_q/LConn1
  vis_roll_horn_q/RConn1 -- vis_roll_horn_q_axisOut/LConn1
  vis_roll_hornT1/RConn1 -- vis_roll_horn_q_axisIn/LConn1
  vis_roll_horn_q_axisOut/RConn1 -- vis_roll_hornT2/LConn1
  vis_roll_hornT2/RConn1 -- vis_roll_servo_horn/RConn1
  vis_roll_horn_in/RConn1 -- vis_roll_horn_q/LConn2
  vis_roll_rod_q_axisIn/RConn1 -- vis_roll_rod_q/LConn1
  vis_roll_rod_q/RConn1 -- vis_roll_rod_q_axisOut/LConn1
  vis_roll_rod_qn_axisIn/RConn1 -- vis_roll_rod_qn/LConn1
  vis_roll_rod_qn/RConn1 -- vis_roll_rod_qn_axisOut/LConn1
  vis_roll_rodT1/RConn1 -- vis_roll_rod_q_axisIn/LConn1
  vis_roll_rod_q_axisOut/RConn1 -- vis_roll_rodT2/LConn1
  vis_roll_rodT2/RConn1 -- vis_roll_rod_qn_axisIn/LConn1
  vis_roll_rod_qn_axisOut/RConn1 -- vis_roll_rodT3/LConn1
  vis_roll_rodT3/RConn1 -- vis_roll_rod/RConn1
  vis_roll_rod_in/RConn1 -- vis_roll_rod_q/LConn2
  vis_roll_rod_inn/RConn1 -- vis_roll_rod_qn/LConn2
  vis_pitch_horn_q_axisIn/RConn1 -- vis_pitch_horn_q/LConn1
  vis_pitch_horn_q/RConn1 -- vis_pitch_horn_q_axisOut/LConn1
  vis_pitch_hornT1/RConn1 -- vis_pitch_horn_q_axisIn/LConn1
  vis_pitch_horn_q_axisOut/RConn1 -- vis_pitch_hornT2/LConn1
  vis_pitch_hornT2/RConn1 -- vis_pitch_servo_horn/RConn1
  vis_pitch_horn_in/RConn1 -- vis_pitch_horn_q/LConn2
  vis_pitch_rod_q_axisIn/RConn1 -- vis_pitch_rod_q/LConn1
  vis_pitch_rod_q/RConn1 -- vis_pitch_rod_q_axisOut/LConn1
  vis_pitch_rod_qn_axisIn/RConn1 -- vis_pitch_rod_qn/LConn1
  vis_pitch_rod_qn/RConn1 -- vis_pitch_rod_qn_axisOut/LConn1
  vis_pitch_rodT1/RConn1 -- vis_pitch_rod_q_axisIn/LConn1
  vis_pitch_rod_q_axisOut/RConn1 -- vis_pitch_rodT2/LConn1
  vis_pitch_rodT2/RConn1 -- vis_pitch_rod_qn_axisIn/LConn1
  vis_pitch_rod_qn_axisOut/RConn1 -- vis_pitch_rodT3/LConn1
  vis_pitch_rodT3/RConn1 -- vis_pitch_rod/RConn1
  vis_pitch_rod_in/RConn1 -- vis_pitch_rod_q/LConn2
  vis_pitch_rod_inn/RConn1 -- vis_pitch_rod_qn/LConn2
